simulink model "rfsoc4x2_ospfb_128"  (R2021a)
settings: Solver=VariableStepAuto  StartTime=0.0  StopTime=2048  RelTol=1e-3
undefined symbols (not defined in the file): pfb_coeff_gen_calc
libraries: xbsIndex_r4 x25898, casper_library_delays x113, casper_library_misc x68, xps_library x1
(part 5 of 221)

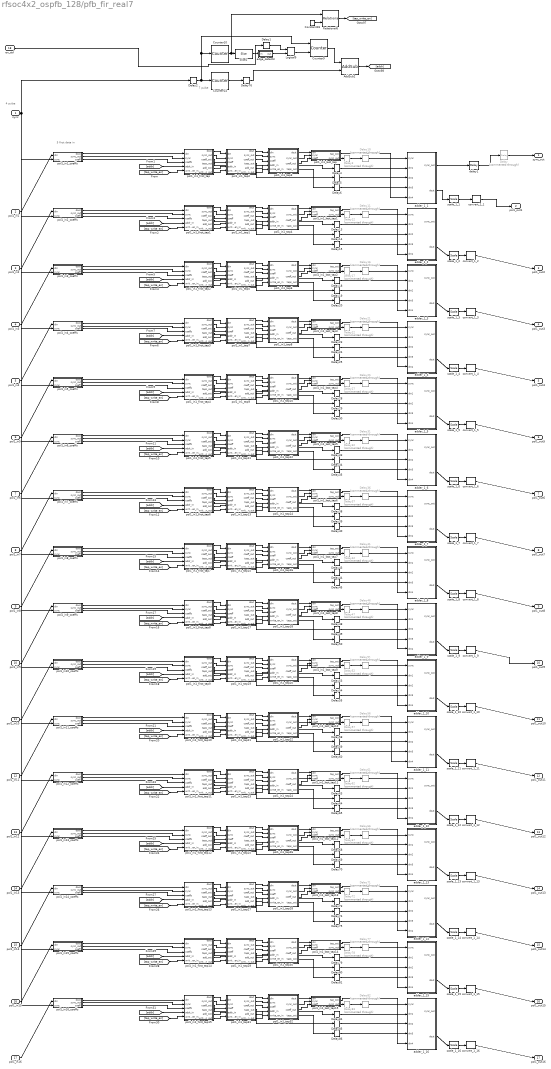
== system rfsoc4x2_ospfb_128/pfb_fir_real7 ==
  note: 5 first data in
  note: 7 pulse
  note: 4 pulse
  sync : Inport
  pol1_in1 : Inport  Port=2
  pol1_in2 : Inport  Port=3
  pol1_in3 : Inport  Port=4
  pol1_in4 : Inport  Port=5
  pol1_in5 : Inport  Port=6
  pol1_in6 : Inport  Port=7
  pol1_in7 : Inport  Port=8
  pol1_in8 : Inport  Port=9
  pol1_in9 : Inport  Port=10
  pol1_in10 : Inport  Port=11
  pol1_in11 : Inport  Port=12
  pol1_in12 : Inport  Port=13
  pol1_in13 : Inport  Port=14
  pol1_in14 : Inport  Port=15
  pol1_in15 : Inport  Port=16
  pol1_in16 : Inport  Port=17
  en_ctrl : Inport  Port=18
  AddSub2 : xbsIndex_r4/AddSub  mode=Addition  use_carryin=off  use_carryout=off  en=off  latency=0  precision=User Defined  arith_type=Unsigned  n_bits=5-1  bin_pt=0  quantization=Truncate  overflow=Wrap  use_behavioral_HDL=off  hw_selection=Fabric  pipelined=off  dbl_ovrd=off  block_type=addsub
  Constant28 : xbsIndex_r4/Constant  const=7  gui_display_data_type=Fixed-point  arith_type=Unsigned  n_bits=log2((2^8 / 2^4))  bin_pt=0  preci_type=Single  exp_width=8  frac_width=24  explicit_period=off  period=1  equ=P=C  opselect=C  inp2=PCIN>>17  opr=+  inp1=P  carry=CIN  dbl_ovrd=off  block_type=constant
  Counter10 : xbsIndex_r4/Counter  cnt_type=Free Running  cnt_to=Inf  operation=Up  start_count=16/2  cnt_by_val=1  arith_type=Unsigned  n_bits=5-1  bin_pt=0  load_pin=off  rst=on  en=off  explicit_period=on  period=1  use_behavioral_HDL=off  implementation=Fabric  dbl_ovrd=off  block_type=counter
  Counter14 : xbsIndex_r4/Counter  cnt_type=Free Running  cnt_to=1023  operation=Up  start_count=0  cnt_by_val=1  arith_type=Unsigned  n_bits=4-1  bin_pt=0  load_pin=off  rst=on  en=off  explicit_period=on  period=1  use_behavioral_HDL=off  implementation=Fabric  dbl_ovrd=off  block_type=counter
  Counter9 : xbsIndex_r4/Counter  cnt_type=Free Running  cnt_to=0  operation=Up  start_count=0  cnt_by_val=16/2  arith_type=Unsigned  n_bits=5-1  bin_pt=0  load_pin=off  rst=on  en=on  explicit_period=on  period=1  use_behavioral_HDL=off  implementation=Fabric  dbl_ovrd=off  block_type=counter
  Delay : xbsIndex_r4/Delay  Commented=through  rst=off  infoeditControl=Selection of Reset will increase slice count due to use of real FFs and instead of SRLs  en=off  latency=47  reg_retiming=off  dbl_ovrd=off  block_type=delay
  Delay1 : xbsIndex_r4/Delay  rst=off  infoeditControl=Selection of Reset will increase slice count due to use of real FFs and instead of SRLs  en=off  latency=4  reg_retiming=off  dbl_ovrd=off  block_type=delay
  Delay{10..11,16,21,26,31,36,41,46,51,56,61,66,71,77,82} (16 alike) : xbsIndex_r4/Delay  Commented=through  rst=off  infoeditControl=Selection of Reset will increase slice count due to use of real FFs and instead of SRLs  en=off  latency=2  reg_retiming=off  dbl_ovrd=off  block_type=delay
  Delay{3,12,17,22,27,32,37,42,47,52,57,62,67,72,78,83} (16 alike) : xbsIndex_r4/Delay  Commented=through  rst=off  infoeditControl=Selection of Reset will increase slice count due to use of real FFs and instead of SRLs  en=off  latency=3  reg_retiming=off  dbl_ovrd=off  block_type=delay
  Delay{2,4,13,18,23,28,33,38,43,48,53,58,63,68,73,79,84} (17 alike) : xbsIndex_r4/Delay  rst=off  infoeditControl=Selection of Reset will increase slice count due to use of real FFs and instead of SRLs  en=off  latency=3  reg_retiming=off  dbl_ovrd=off  block_type=delay
  Delay{5,14,19,24,29,34,39,44,49,54,59,64,69,74,80,85} (16 alike) : xbsIndex_r4/Delay  rst=off  infoeditControl=Selection of Reset will increase slice count due to use of real FFs and instead of SRLs  en=off  latency=2  reg_retiming=off  dbl_ovrd=off  block_type=delay
  Delay{6,15,20,25,30,35,40,45,50,55,60,65,70,75..76,81,86} (17 alike) : xbsIndex_r4/Delay  rst=off  infoeditControl=Selection of Reset will increase slice count due to use of real FFs and instead of SRLs  en=off  latency=1  reg_retiming=off  dbl_ovrd=off  block_type=delay
  Logical9 : xbsIndex_r4/Logical  logical_function=AND  inputs=2  en=off  latency=0  precision=Full  arith_type=Unsigned  n_bits=16  bin_pt=0  align_bp=on  dbl_ovrd=off  block_type=logical
  Relational6 : xbsIndex_r4/Relational  mode=a>b  op_type=Bool  en=off  latency=1  dbl_ovrd=off  block_type=relational
  Slice2 : xbsIndex_r4/Slice  nbits=1  boolean_output=on  mode=Upper Bit Location + Width  bit1=0  base1=MSB of Input  bit0=0  base0=LSB of Input  dbl_ovrd=off  block_type=slice
  adder_1_1 : Subsystem  AncestorBlock=casper_library_misc/adder_tree  mask(adder_tree){n_inputs=4, csp_latency=1, adder_imp=Fabric, first_stage_hdl=on, floating_point=off, dvalid_en=off, float_type=single, frac_width=0, exp_width=0}
      mask prompts: n_inputs "Number of Inputs"; csp_latency "Add Latency"; adder_imp "Adder implementation"; first_stage_hdl "Use behavioural HDL for first stage of adders"; floating_point "floating point"; float_type "float type"; frac_width "fraction length"; exp_width "exponent length"
      mask help:
      | Sums all inputs using a tree of adds and delays.
      |
      | Number of inputs: The number of inputs to the block to be summed
      | Add latency: The number of clock cycles to perform one addition (affects timing)..
      | Adder implementation: choice of fabric or DSP48E core, or behavioral HDL
      | Use behavioural HDL for first stage of adders: Causes the first stage of adders to be absorbed into DSP blocks if multipliers precede them (Virtex 5). Overrides Adder implementation
      mask init:
      | adder_tree_init(gcb, ...
      |     'n_inputs', n_inputs, ...
      |     'csp_latency', csp_latency, ...
      |     'adder_imp', adder_imp, ...
      |     'dvalid_en', dvalid_en, ...
      |     'floating_point', floating_point, ...
      |     'float_type', float_type, ...
      |     'exp_width', exp_width, ...
      |     'frac_width', frac_width, ...     
      |     'first_stage_hdl', first_stage_hdl);
      settings: AttributesFormatString=latency 2
      mask Help: eval('xlWeb(''http://casper.berkeley.edu/wiki/Adder_tree'')')
      mask TypeOptions adder_imp: Behavioral | Fabric | DSP48
      mask Callback floating_point:
      | onoff = get_param(gcb, 'floating_point');
      | if strcmp(onoff,'on')
      |     enable_fixpt = 'off';
      |     set_param_state(gcb, 'float_type', 'on')
      | 
      |     f_type = get_param(gcb, 'float_type');
      |     if strcmp(f_type,'custom')
      |         set_param_state(gcb, 'exp_width', 'on')
      |         set_param_state(gcb, 'frac_width', 'on')
      |     else
      |         set_param_state(gcb, 'exp_width', 'off')
      |         set_param_state(gcb, 'frac_width', 'off')
      |     end
      | 
      | 
      | else
      |     enable_fixpt = 'on';
      |     set_param_state(gcb, 'float_type', 'off')
      |     set_param_state(gcb, 'exp_width', 'off')
      |     set_param_state(gcb, 'frac_width', 'off')
      | end
      mask TypeOptions float_type: single | custom
      mask Callback float_type:
      | f_type = get_param(gcb, 'float_type');
      | if strcmp(f_type,'custom')
      |     set_param_state(gcb, 'exp_width', 'on')
      |     set_param_state(gcb, 'frac_width', 'on')
      | else
      |     set_param_state(gcb, 'exp_width', 'off')
      |     set_param_state(gcb, 'frac_width', 'off')
      | end
  adder_1_10 : Subsystem  AncestorBlock=casper_library_misc/adder_tree  mask(adder_tree){n_inputs=4, csp_latency=1, adder_imp=Fabric, first_stage_hdl=on, floating_point=off, dvalid_en=off, float_type=single, frac_width=0, exp_width=0}
      mask prompts: n_inputs "Number of Inputs"; csp_latency "Add Latency"; adder_imp "Adder implementation"; first_stage_hdl "Use behavioural HDL for first stage of adders"; floating_point "floating point"; float_type "float type"; frac_width "fraction length"; exp_width "exponent length"
      mask help:
      | Sums all inputs using a tree of adds and delays.
      |
      | Number of inputs: The number of inputs to the block to be summed
      | Add latency: The number of clock cycles to perform one addition (affects timing)..
      | Adder implementation: choice of fabric or DSP48E core, or behavioral HDL
      | Use behavioural HDL for first stage of adders: Causes the first stage of adders to be absorbed into DSP blocks if multipliers precede them (Virtex 5). Overrides Adder implementation
      mask init: same as rfsoc4x2_ospfb_128/pfb_fir_real7/adder_1_1
      settings: AttributesFormatString=latency 2
      mask Help: eval('xlWeb(''http://casper.berkeley.edu/wiki/Adder_tree'')')
      mask TypeOptions adder_imp: Behavioral | Fabric | DSP48
      mask Callback floating_point:
      | onoff = get_param(gcb, 'floating_point');
      | if strcmp(onoff,'on')
      |     enable_fixpt = 'off';
      |     set_param_state(gcb, 'float_type', 'on')
      | 
      |     f_type = get_param(gcb, 'float_type');
      |     if strcmp(f_type,'custom')
      |         set_param_state(gcb, 'exp_width', 'on')
      |         set_param_state(gcb, 'frac_width', 'on')
      |     else
      |         set_param_state(gcb, 'exp_width', 'off')
      |         set_param_state(gcb, 'frac_width', 'off')
      |     end
      | 
      | 
      | else
      |     enable_fixpt = 'on';
      |     set_param_state(gcb, 'float_type', 'off')
      |     set_param_state(gcb, 'exp_width', 'off')
      |     set_param_state(gcb, 'frac_width', 'off')
      | end
      mask TypeOptions float_type: single | custom
      mask Callback float_type:
      | f_type = get_param(gcb, 'float_type');
      | if strcmp(f_type,'custom')
      |     set_param_state(gcb, 'exp_width', 'on')
      |     set_param_state(gcb, 'frac_width', 'on')
      | else
      |     set_param_state(gcb, 'exp_width', 'off')
      |     set_param_state(gcb, 'frac_width', 'off')
      | end
  adder_1_11 : Subsystem  AncestorBlock=casper_library_misc/adder_tree  mask(adder_tree){n_inputs=4, csp_latency=1, adder_imp=Fabric, first_stage_hdl=on, floating_point=off, dvalid_en=off, float_type=single, frac_width=0, exp_width=0}
      mask prompts: n_inputs "Number of Inputs"; csp_latency "Add Latency"; adder_imp "Adder implementation"; first_stage_hdl "Use behavioural HDL for first stage of adders"; floating_point "floating point"; float_type "float type"; frac_width "fraction length"; exp_width "exponent length"
      mask help:
      | Sums all inputs using a tree of adds and delays.
      |
      | Number of inputs: The number of inputs to the block to be summed
      | Add latency: The number of clock cycles to perform one addition (affects timing)..
      | Adder implementation: choice of fabric or DSP48E core, or behavioral HDL
      | Use behavioural HDL for first stage of adders: Causes the first stage of adders to be absorbed into DSP blocks if multipliers precede them (Virtex 5). Overrides Adder implementation
      mask init: same as rfsoc4x2_ospfb_128/pfb_fir_real7/adder_1_1
      settings: AttributesFormatString=latency 2
      mask Help: eval('xlWeb(''http://casper.berkeley.edu/wiki/Adder_tree'')')
      mask TypeOptions adder_imp: Behavioral | Fabric | DSP48
      mask Callback floating_point:
      | onoff = get_param(gcb, 'floating_point');
      | if strcmp(onoff,'on')
      |     enable_fixpt = 'off';
      |     set_param_state(gcb, 'float_type', 'on')
      | 
      |     f_type = get_param(gcb, 'float_type');
      |     if strcmp(f_type,'custom')
      |         set_param_state(gcb, 'exp_width', 'on')
      |         set_param_state(gcb, 'frac_width', 'on')
      |     else
      |         set_param_state(gcb, 'exp_width', 'off')
      |         set_param_state(gcb, 'frac_width', 'off')
      |     end
      | 
      | 
      | else
      |     enable_fixpt = 'on';
      |     set_param_state(gcb, 'float_type', 'off')
      |     set_param_state(gcb, 'exp_width', 'off')
      |     set_param_state(gcb, 'frac_width', 'off')
      | end
      mask TypeOptions float_type: single | custom
      mask Callback float_type:
      | f_type = get_param(gcb, 'float_type');
      | if strcmp(f_type,'custom')
      |     set_param_state(gcb, 'exp_width', 'on')
      |     set_param_state(gcb, 'frac_width', 'on')
      | else
      |     set_param_state(gcb, 'exp_width', 'off')
      |     set_param_state(gcb, 'frac_width', 'off')
      | end
  adder_1_12 : Subsystem  AncestorBlock=casper_library_misc/adder_tree  mask(adder_tree){n_inputs=4, csp_latency=1, adder_imp=Fabric, first_stage_hdl=on, floating_point=off, dvalid_en=off, float_type=single, frac_width=0, exp_width=0}
      mask prompts: n_inputs "Number of Inputs"; csp_latency "Add Latency"; adder_imp "Adder implementation"; first_stage_hdl "Use behavioural HDL for first stage of adders"; floating_point "floating point"; float_type "float type"; frac_width "fraction length"; exp_width "exponent length"
      mask help:
      | Sums all inputs using a tree of adds and delays.
      |
      | Number of inputs: The number of inputs to the block to be summed
      | Add latency: The number of clock cycles to perform one addition (affects timing)..
      | Adder implementation: choice of fabric or DSP48E core, or behavioral HDL
      | Use behavioural HDL for first stage of adders: Causes the first stage of adders to be absorbed into DSP blocks if multipliers precede them (Virtex 5). Overrides Adder implementation
      mask init: same as rfsoc4x2_ospfb_128/pfb_fir_real7/adder_1_1
      settings: AttributesFormatString=latency 2
      mask Help: eval('xlWeb(''http://casper.berkeley.edu/wiki/Adder_tree'')')
      mask TypeOptions adder_imp: Behavioral | Fabric | DSP48
      mask Callback floating_point:
      | onoff = get_param(gcb, 'floating_point');
      | if strcmp(onoff,'on')
      |     enable_fixpt = 'off';
      |     set_param_state(gcb, 'float_type', 'on')
      | 
      |     f_type = get_param(gcb, 'float_type');
      |     if strcmp(f_type,'custom')
      |         set_param_state(gcb, 'exp_width', 'on')
      |         set_param_state(gcb, 'frac_width', 'on')
      |     else
      |         set_param_state(gcb, 'exp_width', 'off')
      |         set_param_state(gcb, 'frac_width', 'off')
      |     end
      | 
      | 
      | else
      |     enable_fixpt = 'on';
      |     set_param_state(gcb, 'float_type', 'off')
      |     set_param_state(gcb, 'exp_width', 'off')
      |     set_param_state(gcb, 'frac_width', 'off')
      | end
      mask TypeOptions float_type: single | custom
      mask Callback float_type:
      | f_type = get_param(gcb, 'float_type');
      | if strcmp(f_type,'custom')
      |     set_param_state(gcb, 'exp_width', 'on')
      |     set_param_state(gcb, 'frac_width', 'on')
      | else
      |     set_param_state(gcb, 'exp_width', 'off')
      |     set_param_state(gcb, 'frac_width', 'off')
      | end
  adder_1_13 : Subsystem  AncestorBlock=casper_library_misc/adder_tree  mask(adder_tree){n_inputs=4, csp_latency=1, adder_imp=Fabric, first_stage_hdl=on, floating_point=off, dvalid_en=off, float_type=single, frac_width=0, exp_width=0}
      mask prompts: n_inputs "Number of Inputs"; csp_latency "Add Latency"; adder_imp "Adder implementation"; first_stage_hdl "Use behavioural HDL for first stage of adders"; floating_point "floating point"; float_type "float type"; frac_width "fraction length"; exp_width "exponent length"
      mask help:
      | Sums all inputs using a tree of adds and delays.
      |
      | Number of inputs: The number of inputs to the block to be summed
      | Add latency: The number of clock cycles to perform one addition (affects timing)..
      | Adder implementation: choice of fabric or DSP48E core, or behavioral HDL
      | Use behavioural HDL for first stage of adders: Causes the first stage of adders to be absorbed into DSP blocks if multipliers precede them (Virtex 5). Overrides Adder implementation
      mask init: same as rfsoc4x2_ospfb_128/pfb_fir_real7/adder_1_1
      settings: AttributesFormatString=latency 2
      mask Help: eval('xlWeb(''http://casper.berkeley.edu/wiki/Adder_tree'')')
      mask TypeOptions adder_imp: Behavioral | Fabric | DSP48
      mask Callback floating_point:
      | onoff = get_param(gcb, 'floating_point');
      | if strcmp(onoff,'on')
      |     enable_fixpt = 'off';
      |     set_param_state(gcb, 'float_type', 'on')
      | 
      |     f_type = get_param(gcb, 'float_type');
      |     if strcmp(f_type,'custom')
      |         set_param_state(gcb, 'exp_width', 'on')
      |         set_param_state(gcb, 'frac_width', 'on')
      |     else
      |         set_param_state(gcb, 'exp_width', 'off')
      |         set_param_state(gcb, 'frac_width', 'off')
      |     end
      | 
      | 
      | else
      |     enable_fixpt = 'on';
      |     set_param_state(gcb, 'float_type', 'off')
      |     set_param_state(gcb, 'exp_width', 'off')
      |     set_param_state(gcb, 'frac_width', 'off')
      | end
      mask TypeOptions float_type: single | custom
      mask Callback float_type:
      | f_type = get_param(gcb, 'float_type');
      | if strcmp(f_type,'custom')
      |     set_param_state(gcb, 'exp_width', 'on')
      |     set_param_state(gcb, 'frac_width', 'on')
      | else
      |     set_param_state(gcb, 'exp_width', 'off')
      |     set_param_state(gcb, 'frac_width', 'off')
      | end
  adder_1_14 : Subsystem  AncestorBlock=casper_library_misc/adder_tree  mask(adder_tree){n_inputs=4, csp_latency=1, adder_imp=Fabric, first_stage_hdl=on, floating_point=off, dvalid_en=off, float_type=single, frac_width=0, exp_width=0}
      mask prompts: n_inputs "Number of Inputs"; csp_latency "Add Latency"; adder_imp "Adder implementation"; first_stage_hdl "Use behavioural HDL for first stage of adders"; floating_point "floating point"; float_type "float type"; frac_width "fraction length"; exp_width "exponent length"
      mask help:
      | Sums all inputs using a tree of adds and delays.
      |
      | Number of inputs: The number of inputs to the block to be summed
      | Add latency: The number of clock cycles to perform one addition (affects timing)..
      | Adder implementation: choice of fabric or DSP48E core, or behavioral HDL
      | Use behavioural HDL for first stage of adders: Causes the first stage of adders to be absorbed into DSP blocks if multipliers precede them (Virtex 5). Overrides Adder implementation
      mask init: same as rfsoc4x2_ospfb_128/pfb_fir_real7/adder_1_1
      settings: AttributesFormatString=latency 2
      mask Help: eval('xlWeb(''http://casper.berkeley.edu/wiki/Adder_tree'')')
      mask TypeOptions adder_imp: Behavioral | Fabric | DSP48
      mask Callback floating_point:
      | onoff = get_param(gcb, 'floating_point');
      | if strcmp(onoff,'on')
      |     enable_fixpt = 'off';
      |     set_param_state(gcb, 'float_type', 'on')
      | 
      |     f_type = get_param(gcb, 'float_type');
      |     if strcmp(f_type,'custom')
      |         set_param_state(gcb, 'exp_width', 'on')
      |         set_param_state(gcb, 'frac_width', 'on')
      |     else
      |         set_param_state(gcb, 'exp_width', 'off')
      |         set_param_state(gcb, 'frac_width', 'off')
      |     end
      | 
      | 
      | else
      |     enable_fixpt = 'on';
      |     set_param_state(gcb, 'float_type', 'off')
      |     set_param_state(gcb, 'exp_width', 'off')
      |     set_param_state(gcb, 'frac_width', 'off')
      | end
      mask TypeOptions float_type: single | custom
      mask Callback float_type:
      | f_type = get_param(gcb, 'float_type');
      | if strcmp(f_type,'custom')
      |     set_param_state(gcb, 'exp_width', 'on')
      |     set_param_state(gcb, 'frac_width', 'on')
      | else
      |     set_param_state(gcb, 'exp_width', 'off')
      |     set_param_state(gcb, 'frac_width', 'off')
      | end
  adder_1_15 : Subsystem  AncestorBlock=casper_library_misc/adder_tree  mask(adder_tree){n_inputs=4, csp_latency=1, adder_imp=Fabric, first_stage_hdl=on, floating_point=off, dvalid_en=off, float_type=single, frac_width=0, exp_width=0}
      mask prompts: n_inputs "Number of Inputs"; csp_latency "Add Latency"; adder_imp "Adder implementation"; first_stage_hdl "Use behavioural HDL for first stage of adders"; floating_point "floating point"; float_type "float type"; frac_width "fraction length"; exp_width "exponent length"
      mask help:
      | Sums all inputs using a tree of adds and delays.
      |
      | Number of inputs: The number of inputs to the block to be summed
      | Add latency: The number of clock cycles to perform one addition (affects timing)..
      | Adder implementation: choice of fabric or DSP48E core, or behavioral HDL
      | Use behavioural HDL for first stage of adders: Causes the first stage of adders to be absorbed into DSP blocks if multipliers precede them (Virtex 5). Overrides Adder implementation
      mask init: same as rfsoc4x2_ospfb_128/pfb_fir_real7/adder_1_1
      settings: AttributesFormatString=latency 2
      mask Help: eval('xlWeb(''http://casper.berkeley.edu/wiki/Adder_tree'')')
      mask TypeOptions adder_imp: Behavioral | Fabric | DSP48
      mask Callback floating_point:
      | onoff = get_param(gcb, 'floating_point');
      | if strcmp(onoff,'on')
      |     enable_fixpt = 'off';
      |     set_param_state(gcb, 'float_type', 'on')
      | 
      |     f_type = get_param(gcb, 'float_type');
      |     if strcmp(f_type,'custom')
      |         set_param_state(gcb, 'exp_width', 'on')
      |         set_param_state(gcb, 'frac_width', 'on')
      |     else
      |         set_param_state(gcb, 'exp_width', 'off')
      |         set_param_state(gcb, 'frac_width', 'off')
      |     end
      | 
      | 
      | else
      |     enable_fixpt = 'on';
      |     set_param_state(gcb, 'float_type', 'off')
      |     set_param_state(gcb, 'exp_width', 'off')
      |     set_param_state(gcb, 'frac_width', 'off')
      | end
      mask TypeOptions float_type: single | custom
      mask Callback float_type:
      | f_type = get_param(gcb, 'float_type');
      | if strcmp(f_type,'custom')
      |     set_param_state(gcb, 'exp_width', 'on')
      |     set_param_state(gcb, 'frac_width', 'on')
      | else
      |     set_param_state(gcb, 'exp_width', 'off')
      |     set_param_state(gcb, 'frac_width', 'off')
      | end
  adder_1_16 : Subsystem  AncestorBlock=casper_library_misc/adder_tree  mask(adder_tree){n_inputs=4, csp_latency=1, adder_imp=Fabric, first_stage_hdl=on, floating_point=off, dvalid_en=off, float_type=single, frac_width=0, exp_width=0}
      mask prompts: n_inputs "Number of Inputs"; csp_latency "Add Latency"; adder_imp "Adder implementation"; first_stage_hdl "Use behavioural HDL for first stage of adders"; floating_point "floating point"; float_type "float type"; frac_width "fraction length"; exp_width "exponent length"
      mask help:
      | Sums all inputs using a tree of adds and delays.
      |
      | Number of inputs: The number of inputs to the block to be summed
      | Add latency: The number of clock cycles to perform one addition (affects timing)..
      | Adder implementation: choice of fabric or DSP48E core, or behavioral HDL
      | Use behavioural HDL for first stage of adders: Causes the first stage of adders to be absorbed into DSP blocks if multipliers precede them (Virtex 5). Overrides Adder implementation
      mask init: same as rfsoc4x2_ospfb_128/pfb_fir_real7/adder_1_1
      settings: AttributesFormatString=latency 2
      mask Help: eval('xlWeb(''http://casper.berkeley.edu/wiki/Adder_tree'')')
      mask TypeOptions adder_imp: Behavioral | Fabric | DSP48
      mask Callback floating_point:
      | onoff = get_param(gcb, 'floating_point');
      | if strcmp(onoff,'on')
      |     enable_fixpt = 'off';
      |     set_param_state(gcb, 'float_type', 'on')
      | 
      |     f_type = get_param(gcb, 'float_type');
      |     if strcmp(f_type,'custom')
      |         set_param_state(gcb, 'exp_width', 'on')
      |         set_param_state(gcb, 'frac_width', 'on')
      |     else
      |         set_param_state(gcb, 'exp_width', 'off')
      |         set_param_state(gcb, 'frac_width', 'off')
      |     end
      | 
      | 
      | else
      |     enable_fixpt = 'on';
      |     set_param_state(gcb, 'float_type', 'off')
      |     set_param_state(gcb, 'exp_width', 'off')
      |     set_param_state(gcb, 'frac_width', 'off')
      | end
      mask TypeOptions float_type: single | custom
      mask Callback float_type:
      | f_type = get_param(gcb, 'float_type');
      | if strcmp(f_type,'custom')
      |     set_param_state(gcb, 'exp_width', 'on')
      |     set_param_state(gcb, 'frac_width', 'on')
      | else
      |     set_param_state(gcb, 'exp_width', 'off')
      |     set_param_state(gcb, 'frac_width', 'off')
      | end
  adder_1_2 : Subsystem  AncestorBlock=casper_library_misc/adder_tree  mask(adder_tree){n_inputs=4, csp_latency=1, adder_imp=Fabric, first_stage_hdl=on, floating_point=off, dvalid_en=off, float_type=single, frac_width=0, exp_width=0}
      mask prompts: n_inputs "Number of Inputs"; csp_latency "Add Latency"; adder_imp "Adder implementation"; first_stage_hdl "Use behavioural HDL for first stage of adders"; floating_point "floating point"; float_type "float type"; frac_width "fraction length"; exp_width "exponent length"
      mask help:
      | Sums all inputs using a tree of adds and delays.
      |
      | Number of inputs: The number of inputs to the block to be summed
      | Add latency: The number of clock cycles to perform one addition (affects timing)..
      | Adder implementation: choice of fabric or DSP48E core, or behavioral HDL
      | Use behavioural HDL for first stage of adders: Causes the first stage of adders to be absorbed into DSP blocks if multipliers precede them (Virtex 5). Overrides Adder implementation
      mask init: same as rfsoc4x2_ospfb_128/pfb_fir_real7/adder_1_1
      settings: AttributesFormatString=latency 2
      mask Help: eval('xlWeb(''http://casper.berkeley.edu/wiki/Adder_tree'')')
      mask TypeOptions adder_imp: Behavioral | Fabric | DSP48
      mask Callback floating_point:
      | onoff = get_param(gcb, 'floating_point');
      | if strcmp(onoff,'on')
      |     enable_fixpt = 'off';
      |     set_param_state(gcb, 'float_type', 'on')
      | 
      |     f_type = get_param(gcb, 'float_type');
      |     if strcmp(f_type,'custom')
      |         set_param_state(gcb, 'exp_width', 'on')
      |         set_param_state(gcb, 'frac_width', 'on')
      |     else
      |         set_param_state(gcb, 'exp_width', 'off')
      |         set_param_state(gcb, 'frac_width', 'off')
      |     end
      | 
      | 
      | else
      |     enable_fixpt = 'on';
      |     set_param_state(gcb, 'float_type', 'off')
      |     set_param_state(gcb, 'exp_width', 'off')
      |     set_param_state(gcb, 'frac_width', 'off')
      | end
      mask TypeOptions float_type: single | custom
      mask Callback float_type:
      | f_type = get_param(gcb, 'float_type');
      | if strcmp(f_type,'custom')
      |     set_param_state(gcb, 'exp_width', 'on')
      |     set_param_state(gcb, 'frac_width', 'on')
      | else
      |     set_param_state(gcb, 'exp_width', 'off')
      |     set_param_state(gcb, 'frac_width', 'off')
      | end
  adder_1_3 : Subsystem  AncestorBlock=casper_library_misc/adder_tree  mask(adder_tree){n_inputs=4, csp_latency=1, adder_imp=Fabric, first_stage_hdl=on, floating_point=off, dvalid_en=off, float_type=single, frac_width=0, exp_width=0}
      mask prompts: n_inputs "Number of Inputs"; csp_latency "Add Latency"; adder_imp "Adder implementation"; first_stage_hdl "Use behavioural HDL for first stage of adders"; floating_point "floating point"; float_type "float type"; frac_width "fraction length"; exp_width "exponent length"
      mask help:
      | Sums all inputs using a tree of adds and delays.
      |
      | Number of inputs: The number of inputs to the block to be summed
      | Add latency: The number of clock cycles to perform one addition (affects timing)..
      | Adder implementation: choice of fabric or DSP48E core, or behavioral HDL
      | Use behavioural HDL for first stage of adders: Causes the first stage of adders to be absorbed into DSP blocks if multipliers precede them (Virtex 5). Overrides Adder implementation
      mask init: same as rfsoc4x2_ospfb_128/pfb_fir_real7/adder_1_1
      settings: AttributesFormatString=latency 2
      mask Help: eval('xlWeb(''http://casper.berkeley.edu/wiki/Adder_tree'')')
      mask TypeOptions adder_imp: Behavioral | Fabric | DSP48
      mask Callback floating_point:
      | onoff = get_param(gcb, 'floating_point');
      | if strcmp(onoff,'on')
      |     enable_fixpt = 'off';
      |     set_param_state(gcb, 'float_type', 'on')
      | 
      |     f_type = get_param(gcb, 'float_type');
      |     if strcmp(f_type,'custom')
      |         set_param_state(gcb, 'exp_width', 'on')
      |         set_param_state(gcb, 'frac_width', 'on')
      |     else
      |         set_param_state(gcb, 'exp_width', 'off')
      |         set_param_state(gcb, 'frac_width', 'off')
      |     end
      | 
      | 
      | else
      |     enable_fixpt = 'on';
      |     set_param_state(gcb, 'float_type', 'off')
      |     set_param_state(gcb, 'exp_width', 'off')
      |     set_param_state(gcb, 'frac_width', 'off')
      | end
      mask TypeOptions float_type: single | custom
      mask Callback float_type:
      | f_type = get_param(gcb, 'float_type');
      | if strcmp(f_type,'custom')
      |     set_param_state(gcb, 'exp_width', 'on')
      |     set_param_state(gcb, 'frac_width', 'on')
      | else
      |     set_param_state(gcb, 'exp_width', 'off')
      |     set_param_state(gcb, 'frac_width', 'off')
      | end
  adder_1_4 : Subsystem  AncestorBlock=casper_library_misc/adder_tree  mask(adder_tree){n_inputs=4, csp_latency=1, adder_imp=Fabric, first_stage_hdl=on, floating_point=off, dvalid_en=off, float_type=single, frac_width=0, exp_width=0}
      mask prompts: n_inputs "Number of Inputs"; csp_latency "Add Latency"; adder_imp "Adder implementation"; first_stage_hdl "Use behavioural HDL for first stage of adders"; floating_point "floating point"; float_type "float type"; frac_width "fraction length"; exp_width "exponent length"
      mask help:
      | Sums all inputs using a tree of adds and delays.
      |
      | Number of inputs: The number of inputs to the block to be summed
      | Add latency: The number of clock cycles to perform one addition (affects timing)..
      | Adder implementation: choice of fabric or DSP48E core, or behavioral HDL
      | Use behavioural HDL for first stage of adders: Causes the first stage of adders to be absorbed into DSP blocks if multipliers precede them (Virtex 5). Overrides Adder implementation
      mask init: same as rfsoc4x2_ospfb_128/pfb_fir_real7/adder_1_1
      settings: AttributesFormatString=latency 2
      mask Help: eval('xlWeb(''http://casper.berkeley.edu/wiki/Adder_tree'')')
      mask TypeOptions adder_imp: Behavioral | Fabric | DSP48
      mask Callback floating_point:
      | onoff = get_param(gcb, 'floating_point');
      | if strcmp(onoff,'on')
      |     enable_fixpt = 'off';
      |     set_param_state(gcb, 'float_type', 'on')
      | 
      |     f_type = get_param(gcb, 'float_type');
      |     if strcmp(f_type,'custom')
      |         set_param_state(gcb, 'exp_width', 'on')
      |         set_param_state(gcb, 'frac_width', 'on')
      |     else
      |         set_param_state(gcb, 'exp_width', 'off')
      |         set_param_state(gcb, 'frac_width', 'off')
      |     end
      | 
      | 
      | else
      |     enable_fixpt = 'on';
      |     set_param_state(gcb, 'float_type', 'off')
      |     set_param_state(gcb, 'exp_width', 'off')
      |     set_param_state(gcb, 'frac_width', 'off')
      | end
      mask TypeOptions float_type: single | custom
      mask Callback float_type:
      | f_type = get_param(gcb, 'float_type');
      | if strcmp(f_type,'custom')
      |     set_param_state(gcb, 'exp_width', 'on')
      |     set_param_state(gcb, 'frac_width', 'on')
      | else
      |     set_param_state(gcb, 'exp_width', 'off')
      |     set_param_state(gcb, 'frac_width', 'off')
      | end
  adder_1_5 : Subsystem  AncestorBlock=casper_library_misc/adder_tree  mask(adder_tree){n_inputs=4, csp_latency=1, adder_imp=Fabric, first_stage_hdl=on, floating_point=off, dvalid_en=off, float_type=single, frac_width=0, exp_width=0}
      mask prompts: n_inputs "Number of Inputs"; csp_latency "Add Latency"; adder_imp "Adder implementation"; first_stage_hdl "Use behavioural HDL for first stage of adders"; floating_point "floating point"; float_type "float type"; frac_width "fraction length"; exp_width "exponent length"
      mask help:
      | Sums all inputs using a tree of adds and delays.
      |
      | Number of inputs: The number of inputs to the block to be summed
      | Add latency: The number of clock cycles to perform one addition (affects timing)..
      | Adder implementation: choice of fabric or DSP48E core, or behavioral HDL
      | Use behavioural HDL for first stage of adders: Causes the first stage of adders to be absorbed into DSP blocks if multipliers precede them (Virtex 5). Overrides Adder implementation
      mask init: same as rfsoc4x2_ospfb_128/pfb_fir_real7/adder_1_1
      settings: AttributesFormatString=latency 2
      mask Help: eval('xlWeb(''http://casper.berkeley.edu/wiki/Adder_tree'')')
      mask TypeOptions adder_imp: Behavioral | Fabric | DSP48
      mask Callback floating_point:
      | onoff = get_param(gcb, 'floating_point');
      | if strcmp(onoff,'on')
      |     enable_fixpt = 'off';
      |     set_param_state(gcb, 'float_type', 'on')
      | 
      |     f_type = get_param(gcb, 'float_type');
      |     if strcmp(f_type,'custom')
      |         set_param_state(gcb, 'exp_width', 'on')
      |         set_param_state(gcb, 'frac_width', 'on')
      |     else
      |         set_param_state(gcb, 'exp_width', 'off')
      |         set_param_state(gcb, 'frac_width', 'off')
      |     end
      | 
      | 
      | else
      |     enable_fixpt = 'on';
      |     set_param_state(gcb, 'float_type', 'off')
      |     set_param_state(gcb, 'exp_width', 'off')
      |     set_param_state(gcb, 'frac_width', 'off')
      | end
      mask TypeOptions float_type: single | custom
      mask Callback float_type:
      | f_type = get_param(gcb, 'float_type');
      | if strcmp(f_type,'custom')
      |     set_param_state(gcb, 'exp_width', 'on')
      |     set_param_state(gcb, 'frac_width', 'on')
      | else
      |     set_param_state(gcb, 'exp_width', 'off')
      |     set_param_state(gcb, 'frac_width', 'off')
      | end
  adder_1_6 : Subsystem  AncestorBlock=casper_library_misc/adder_tree  mask(adder_tree){n_inputs=4, csp_latency=1, adder_imp=Fabric, first_stage_hdl=on, floating_point=off, dvalid_en=off, float_type=single, frac_width=0, exp_width=0}
      mask prompts: n_inputs "Number of Inputs"; csp_latency "Add Latency"; adder_imp "Adder implementation"; first_stage_hdl "Use behavioural HDL for first stage of adders"; floating_point "floating point"; float_type "float type"; frac_width "fraction length"; exp_width "exponent length"
      mask help:
      | Sums all inputs using a tree of adds and delays.
      |
      | Number of inputs: The number of inputs to the block to be summed
      | Add latency: The number of clock cycles to perform one addition (affects timing)..
      | Adder implementation: choice of fabric or DSP48E core, or behavioral HDL
      | Use behavioural HDL for first stage of adders: Causes the first stage of adders to be absorbed into DSP blocks if multipliers precede them (Virtex 5). Overrides Adder implementation
      mask init: same as rfsoc4x2_ospfb_128/pfb_fir_real7/adder_1_1
      settings: AttributesFormatString=latency 2
      mask Help: eval('xlWeb(''http://casper.berkeley.edu/wiki/Adder_tree'')')
      mask TypeOptions adder_imp: Behavioral | Fabric | DSP48
      mask Callback floating_point:
      | onoff = get_param(gcb, 'floating_point');
      | if strcmp(onoff,'on')
      |     enable_fixpt = 'off';
      |     set_param_state(gcb, 'float_type', 'on')
      | 
      |     f_type = get_param(gcb, 'float_type');
      |     if strcmp(f_type,'custom')
      |         set_param_state(gcb, 'exp_width', 'on')
      |         set_param_state(gcb, 'frac_width', 'on')
      |     else
      |         set_param_state(gcb, 'exp_width', 'off')
      |         set_param_state(gcb, 'frac_width', 'off')
      |     end
      | 
      | 
      | else
      |     enable_fixpt = 'on';
      |     set_param_state(gcb, 'float_type', 'off')
      |     set_param_state(gcb, 'exp_width', 'off')
      |     set_param_state(gcb, 'frac_width', 'off')
      | end
      mask TypeOptions float_type: single | custom
      mask Callback float_type:
      | f_type = get_param(gcb, 'float_type');
      | if strcmp(f_type,'custom')
      |     set_param_state(gcb, 'exp_width', 'on')
      |     set_param_state(gcb, 'frac_width', 'on')
      | else
      |     set_param_state(gcb, 'exp_width', 'off')
      |     set_param_state(gcb, 'frac_width', 'off')
      | end
  adder_1_7 : Subsystem  AncestorBlock=casper_library_misc/adder_tree  mask(adder_tree){n_inputs=4, csp_latency=1, adder_imp=Fabric, first_stage_hdl=on, floating_point=off, dvalid_en=off, float_type=single, frac_width=0, exp_width=0}
      mask prompts: n_inputs "Number of Inputs"; csp_latency "Add Latency"; adder_imp "Adder implementation"; first_stage_hdl "Use behavioural HDL for first stage of adders"; floating_point "floating point"; float_type "float type"; frac_width "fraction length"; exp_width "exponent length"
      mask help:
      | Sums all inputs using a tree of adds and delays.
      |
      | Number of inputs: The number of inputs to the block to be summed
      | Add latency: The number of clock cycles to perform one addition (affects timing)..
      | Adder implementation: choice of fabric or DSP48E core, or behavioral HDL
      | Use behavioural HDL for first stage of adders: Causes the first stage of adders to be absorbed into DSP blocks if multipliers precede them (Virtex 5). Overrides Adder implementation
      mask init: same as rfsoc4x2_ospfb_128/pfb_fir_real7/adder_1_1
      settings: AttributesFormatString=latency 2
      mask Help: eval('xlWeb(''http://casper.berkeley.edu/wiki/Adder_tree'')')
      mask TypeOptions adder_imp: Behavioral | Fabric | DSP48
      mask Callback floating_point:
      | onoff = get_param(gcb, 'floating_point');
      | if strcmp(onoff,'on')
      |     enable_fixpt = 'off';
      |     set_param_state(gcb, 'float_type', 'on')
      | 
      |     f_type = get_param(gcb, 'float_type');
      |     if strcmp(f_type,'custom')
      |         set_param_state(gcb, 'exp_width', 'on')
      |         set_param_state(gcb, 'frac_width', 'on')
      |     else
      |         set_param_state(gcb, 'exp_width', 'off')
      |         set_param_state(gcb, 'frac_width', 'off')
      |     end
      | 
      | 
      | else
      |     enable_fixpt = 'on';
      |     set_param_state(gcb, 'float_type', 'off')
      |     set_param_state(gcb, 'exp_width', 'off')
      |     set_param_state(gcb, 'frac_width', 'off')
      | end
      mask TypeOptions float_type: single | custom
      mask Callback float_type:
      | f_type = get_param(gcb, 'float_type');
      | if strcmp(f_type,'custom')
      |     set_param_state(gcb, 'exp_width', 'on')
      |     set_param_state(gcb, 'frac_width', 'on')
      | else
      |     set_param_state(gcb, 'exp_width', 'off')
      |     set_param_state(gcb, 'frac_width', 'off')
      | end
  adder_1_8 : Subsystem  AncestorBlock=casper_library_misc/adder_tree  mask(adder_tree){n_inputs=4, csp_latency=1, adder_imp=Fabric, first_stage_hdl=on, floating_point=off, dvalid_en=off, float_type=single, frac_width=0, exp_width=0}
      mask prompts: n_inputs "Number of Inputs"; csp_latency "Add Latency"; adder_imp "Adder implementation"; first_stage_hdl "Use behavioural HDL for first stage of adders"; floating_point "floating point"; float_type "float type"; frac_width "fraction length"; exp_width "exponent length"
      mask help:
      | Sums all inputs using a tree of adds and delays.
      |
      | Number of inputs: The number of inputs to the block to be summed
      | Add latency: The number of clock cycles to perform one addition (affects timing)..
      | Adder implementation: choice of fabric or DSP48E core, or behavioral HDL
      | Use behavioural HDL for first stage of adders: Causes the first stage of adders to be absorbed into DSP blocks if multipliers precede them (Virtex 5). Overrides Adder implementation
      mask init: same as rfsoc4x2_ospfb_128/pfb_fir_real7/adder_1_1
      settings: AttributesFormatString=latency 2
      mask Help: eval('xlWeb(''http://casper.berkeley.edu/wiki/Adder_tree'')')
      mask TypeOptions adder_imp: Behavioral | Fabric | DSP48
      mask Callback floating_point:
      | onoff = get_param(gcb, 'floating_point');
      | if strcmp(onoff,'on')
      |     enable_fixpt = 'off';
      |     set_param_state(gcb, 'float_type', 'on')
      | 
      |     f_type = get_param(gcb, 'float_type');
      |     if strcmp(f_type,'custom')
      |         set_param_state(gcb, 'exp_width', 'on')
      |         set_param_state(gcb, 'frac_width', 'on')
      |     else
      |         set_param_state(gcb, 'exp_width', 'off')
      |         set_param_state(gcb, 'frac_width', 'off')
      |     end
      | 
      | 
      | else
      |     enable_fixpt = 'on';
      |     set_param_state(gcb, 'float_type', 'off')
      |     set_param_state(gcb, 'exp_width', 'off')
      |     set_param_state(gcb, 'frac_width', 'off')
      | end
      mask TypeOptions float_type: single | custom
      mask Callback float_type:
      | f_type = get_param(gcb, 'float_type');
      | if strcmp(f_type,'custom')
      |     set_param_state(gcb, 'exp_width', 'on')
      |     set_param_state(gcb, 'frac_width', 'on')
      | else
      |     set_param_state(gcb, 'exp_width', 'off')
      |     set_param_state(gcb, 'frac_width', 'off')
      | end
  adder_1_9 : Subsystem  AncestorBlock=casper_library_misc/adder_tree  mask(adder_tree){n_inputs=4, csp_latency=1, adder_imp=Fabric, first_stage_hdl=on, floating_point=off, dvalid_en=off, float_type=single, frac_width=0, exp_width=0}
      mask prompts: n_inputs "Number of Inputs"; csp_latency "Add Latency"; adder_imp "Adder implementation"; first_stage_hdl "Use behavioural HDL for first stage of adders"; floating_point "floating point"; float_type "float type"; frac_width "fraction length"; exp_width "exponent length"
      mask help:
      | Sums all inputs using a tree of adds and delays.
      |
      | Number of inputs: The number of inputs to the block to be summed
      | Add latency: The number of clock cycles to perform one addition (affects timing)..
      | Adder implementation: choice of fabric or DSP48E core, or behavioral HDL
      | Use behavioural HDL for first stage of adders: Causes the first stage of adders to be absorbed into DSP blocks if multipliers precede them (Virtex 5). Overrides Adder implementation
      mask init: same as rfsoc4x2_ospfb_128/pfb_fir_real7/adder_1_1
      settings: AttributesFormatString=latency 2
      mask Help: eval('xlWeb(''http://casper.berkeley.edu/wiki/Adder_tree'')')
      mask TypeOptions adder_imp: Behavioral | Fabric | DSP48
      mask Callback floating_point:
      | onoff = get_param(gcb, 'floating_point');
      | if strcmp(onoff,'on')
      |     enable_fixpt = 'off';
      |     set_param_state(gcb, 'float_type', 'on')
      | 
      |     f_type = get_param(gcb, 'float_type');
      |     if strcmp(f_type,'custom')
      |         set_param_state(gcb, 'exp_width', 'on')
      |         set_param_state(gcb, 'frac_width', 'on')
      |     else
      |         set_param_state(gcb, 'exp_width', 'off')
      |         set_param_state(gcb, 'frac_width', 'off')
      |     end
      | 
      | 
      | else
      |     enable_fixpt = 'on';
      |     set_param_state(gcb, 'float_type', 'off')
      |     set_param_state(gcb, 'exp_width', 'off')
      |     set_param_state(gcb, 'frac_width', 'off')
      | end
      mask TypeOptions float_type: single | custom
      mask Callback float_type:
      | f_type = get_param(gcb, 'float_type');
      | if strcmp(f_type,'custom')
      |     set_param_state(gcb, 'exp_width', 'on')
      |     set_param_state(gcb, 'frac_width', 'on')
      | else
      |     set_param_state(gcb, 'exp_width', 'off')
      |     set_param_state(gcb, 'frac_width', 'off')
      | end
  convert_1_{1..16} (16 alike) : xbsIndex_r4/Convert  gui_display_data_type=Fixed-point  arith_type="Signed  (2's comp)"  n_bits=18  bin_pt=17  float_type=Single  exp_bits=8  fraction_bits=24  quantization="Round  (unbiased: Even Values)"  overflow=Wrap  en=off  latency=1  pipeline=on  dbl_ovrd=off  block_type=convert
  delay1 : xbsIndex_r4/Delay  rst=off  infoeditControl=Selection of Reset will increase slice count due to use of real FFs and instead of SRLs  en=off  latency=1  reg_retiming=off  dbl_ovrd=off  block_type=delay
  edge_detect3 : Subsystem  AncestorBlock=casper_library_misc/edge_detect  mask(edge_detect){edge=Falling, polarity=Active High, x_in=[0 0.08 0.08 0.16 0.16 0.24 0.24 0.32 0.32 0.4], y_in=[-1 -1  1  1  1  1  1  1  1  1], x_out=[0.6 0.68 0.68 0.76 0.76 0.84 0.84 0.92 0.92 1], y_out=[-1 -1  1  1 -1 -1 -1 -1 -1 -1]}
      mask prompts: edge "Edge Type"; polarity "Output Polarity"; x_in "Input X Positions"; y_in "Input Y Positions"; x_out "Output X Positions"; y_out "Output Y Positions"
      mask help: Output is active for one-cycle after each edge of the specified type (i.e. rising, falling or both).
      mask init: same as rfsoc4x2_ospfb_128/edge_detect1
      settings: AttributesFormatString=|
      | falling edges
      | active high
      mask Help: Output is active for one-cycle after each edge of the specified type (i.e. rising, falling, or both).  Latency is zero.
      mask TypeOptions edge: Rising | Falling | Both
      mask TypeOptions polarity: Active High | Active Low
      mask Display:
      | plot(x_in_num,0.5+y_in_num*0.2);
      | plot(x_out_num,0.5+y_out_num*0.2);
  pol1_in10_coeffs : Subsystem  AncestorBlock=casper_library_pfbs/pfb_coeff_gen  mask(pfb_coeff_gen){PFBSize=8, CoeffBitWidth=16, TotalTaps=4, CoeffDistMem=off, WindowType=hamming, bram_latency=2, n_inputs=4, nput=9, fwidth=2, debug_mode=off, fan_latency=1}
      mask prompts: PFBSize "Size of PFB: (2^? pnts)"; CoeffBitWidth "Bitwidth of Coefficients:"; TotalTaps "Total Number of Taps:"; CoeffDistMem "Implement Coeff Gen in Distributed Memory"; WindowType "Windowing Function:"; bram_latency "BRAM Latency"; n_inputs "Number of Simultaneous Inputs: (2^?)"; nput "This is input number:"; fwidth "Bin Width (normal=1)"; debug_mode "Debug mode - coeffs are a [1:pfb_size*taps] ramp."; fan_latency "Fanout latency"
      mask init:
      | pfb_coeff_gen_init(gcb, ...
      |     'PFBSize', PFBSize, ...
      |     'CoeffBitWidth', CoeffBitWidth, ...
      |     'TotalTaps', TotalTaps, ...
      |     'CoeffDistMem', CoeffDistMem, ...
      |     'WindowType', WindowType, ...
      |     'bram_latency', bram_latency, ...
      |     'n_inputs', n_inputs, ...
      |     'nput', nput, ...
      |     'fwidth', fwidth, ...
      |     'fan_latency', fan_latency, ...
      |     'debug_mode', debug_mode);
      settings: AttributesFormatString=|
      | PFBSize=8, n_inputs=4,
      | taps=4, input=9
  pol1_in11_coeffs : Subsystem  AncestorBlock=casper_library_pfbs/pfb_coeff_gen  mask(pfb_coeff_gen){PFBSize=8, CoeffBitWidth=16, TotalTaps=4, CoeffDistMem=off, WindowType=hamming, bram_latency=2, n_inputs=4, nput=10, fwidth=2, debug_mode=off, fan_latency=1}
      mask prompts: PFBSize "Size of PFB: (2^? pnts)"; CoeffBitWidth "Bitwidth of Coefficients:"; TotalTaps "Total Number of Taps:"; CoeffDistMem "Implement Coeff Gen in Distributed Memory"; WindowType "Windowing Function:"; bram_latency "BRAM Latency"; n_inputs "Number of Simultaneous Inputs: (2^?)"; nput "This is input number:"; fwidth "Bin Width (normal=1)"; debug_mode "Debug mode - coeffs are a [1:pfb_size*taps] ramp."; fan_latency "Fanout latency"
      mask init: same as rfsoc4x2_ospfb_128/pfb_fir_real7/pol1_in10_coeffs
      settings: AttributesFormatString=|
      | PFBSize=8, n_inputs=4,
      | taps=4, input=10
  pol1_in12_coeffs : Subsystem  AncestorBlock=casper_library_pfbs/pfb_coeff_gen  mask(pfb_coeff_gen){PFBSize=8, CoeffBitWidth=16, TotalTaps=4, CoeffDistMem=off, WindowType=hamming, bram_latency=2, n_inputs=4, nput=11, fwidth=2, debug_mode=off, fan_latency=1}
      mask prompts: PFBSize "Size of PFB: (2^? pnts)"; CoeffBitWidth "Bitwidth of Coefficients:"; TotalTaps "Total Number of Taps:"; CoeffDistMem "Implement Coeff Gen in Distributed Memory"; WindowType "Windowing Function:"; bram_latency "BRAM Latency"; n_inputs "Number of Simultaneous Inputs: (2^?)"; nput "This is input number:"; fwidth "Bin Width (normal=1)"; debug_mode "Debug mode - coeffs are a [1:pfb_size*taps] ramp."; fan_latency "Fanout latency"
      mask init: same as rfsoc4x2_ospfb_128/pfb_fir_real7/pol1_in10_coeffs
      settings: AttributesFormatString=|
      | PFBSize=8, n_inputs=4,
      | taps=4, input=11
  pol1_in13_coeffs : Subsystem  AncestorBlock=casper_library_pfbs/pfb_coeff_gen  mask(pfb_coeff_gen){PFBSize=8, CoeffBitWidth=16, TotalTaps=4, CoeffDistMem=off, WindowType=hamming, bram_latency=2, n_inputs=4, nput=12, fwidth=2, debug_mode=off, fan_latency=1}
      mask prompts: PFBSize "Size of PFB: (2^? pnts)"; CoeffBitWidth "Bitwidth of Coefficients:"; TotalTaps "Total Number of Taps:"; CoeffDistMem "Implement Coeff Gen in Distributed Memory"; WindowType "Windowing Function:"; bram_latency "BRAM Latency"; n_inputs "Number of Simultaneous Inputs: (2^?)"; nput "This is input number:"; fwidth "Bin Width (normal=1)"; debug_mode "Debug mode - coeffs are a [1:pfb_size*taps] ramp."; fan_latency "Fanout latency"
      mask init: same as rfsoc4x2_ospfb_128/pfb_fir_real7/pol1_in10_coeffs
      settings: AttributesFormatString=|
      | PFBSize=8, n_inputs=4,
      | taps=4, input=12
  pol1_in14_coeffs : Subsystem  AncestorBlock=casper_library_pfbs/pfb_coeff_gen  mask(pfb_coeff_gen){PFBSize=8, CoeffBitWidth=16, TotalTaps=4, CoeffDistMem=off, WindowType=hamming, bram_latency=2, n_inputs=4, nput=13, fwidth=2, debug_mode=off, fan_latency=1}
      mask prompts: PFBSize "Size of PFB: (2^? pnts)"; CoeffBitWidth "Bitwidth of Coefficients:"; TotalTaps "Total Number of Taps:"; CoeffDistMem "Implement Coeff Gen in Distributed Memory"; WindowType "Windowing Function:"; bram_latency "BRAM Latency"; n_inputs "Number of Simultaneous Inputs: (2^?)"; nput "This is input number:"; fwidth "Bin Width (normal=1)"; debug_mode "Debug mode - coeffs are a [1:pfb_size*taps] ramp."; fan_latency "Fanout latency"
      mask init: same as rfsoc4x2_ospfb_128/pfb_fir_real7/pol1_in10_coeffs
      settings: AttributesFormatString=|
      | PFBSize=8, n_inputs=4,
      | taps=4, input=13
  pol1_in15_coeffs : Subsystem  AncestorBlock=casper_library_pfbs/pfb_coeff_gen  mask(pfb_coeff_gen){PFBSize=8, CoeffBitWidth=16, TotalTaps=4, CoeffDistMem=off, WindowType=hamming, bram_latency=2, n_inputs=4, nput=14, fwidth=2, debug_mode=off, fan_latency=1}
      mask prompts: PFBSize "Size of PFB: (2^? pnts)"; CoeffBitWidth "Bitwidth of Coefficients:"; TotalTaps "Total Number of Taps:"; CoeffDistMem "Implement Coeff Gen in Distributed Memory"; WindowType "Windowing Function:"; bram_latency "BRAM Latency"; n_inputs "Number of Simultaneous Inputs: (2^?)"; nput "This is input number:"; fwidth "Bin Width (normal=1)"; debug_mode "Debug mode - coeffs are a [1:pfb_size*taps] ramp."; fan_latency "Fanout latency"
      mask init: same as rfsoc4x2_ospfb_128/pfb_fir_real7/pol1_in10_coeffs
      settings: AttributesFormatString=|
      | PFBSize=8, n_inputs=4,
      | taps=4, input=14
  pol1_in16_coeffs : Subsystem  AncestorBlock=casper_library_pfbs/pfb_coeff_gen  mask(pfb_coeff_gen){PFBSize=8, CoeffBitWidth=16, TotalTaps=4, CoeffDistMem=off, WindowType=hamming, bram_latency=2, n_inputs=4, nput=15, fwidth=2, debug_mode=off, fan_latency=1}
      mask prompts: PFBSize "Size of PFB: (2^? pnts)"; CoeffBitWidth "Bitwidth of Coefficients:"; TotalTaps "Total Number of Taps:"; CoeffDistMem "Implement Coeff Gen in Distributed Memory"; WindowType "Windowing Function:"; bram_latency "BRAM Latency"; n_inputs "Number of Simultaneous Inputs: (2^?)"; nput "This is input number:"; fwidth "Bin Width (normal=1)"; debug_mode "Debug mode - coeffs are a [1:pfb_size*taps] ramp."; fan_latency "Fanout latency"
      mask init: same as rfsoc4x2_ospfb_128/pfb_fir_real7/pol1_in10_coeffs
      settings: AttributesFormatString=|
      | PFBSize=8, n_inputs=4,
      | taps=4, input=15
  pol1_in1_coeffs : Subsystem  AncestorBlock=casper_library_pfbs/pfb_coeff_gen  mask(pfb_coeff_gen){PFBSize=8, CoeffBitWidth=16, TotalTaps=4, CoeffDistMem=off, WindowType=hamming, bram_latency=2, n_inputs=4, nput=0, fwidth=2, debug_mode=off, fan_latency=1}
      mask prompts: PFBSize "Size of PFB: (2^? pnts)"; CoeffBitWidth "Bitwidth of Coefficients:"; TotalTaps "Total Number of Taps:"; CoeffDistMem "Implement Coeff Gen in Distributed Memory"; WindowType "Windowing Function:"; bram_latency "BRAM Latency"; n_inputs "Number of Simultaneous Inputs: (2^?)"; nput "This is input number:"; fwidth "Bin Width (normal=1)"; debug_mode "Debug mode - coeffs are a [1:pfb_size*taps] ramp."; fan_latency "Fanout latency"
      mask init: same as rfsoc4x2_ospfb_128/pfb_fir_real7/pol1_in10_coeffs
      settings: AttributesFormatString=|
      | PFBSize=8, n_inputs=4,
      | taps=4, input=0
  pol1_in1_first_tap : Subsystem  AncestorBlock=casper_library_pfbs/first_tap_real  mask(first_tap_real){PFBSize=8, n_pol_blocks=1, CoeffBitWidth=16, TotalTaps=4, BitWidthIn=16, WindowType=hamming, mult_latency=2, bram_latency=2, n_inputs=4, fwidth=2, use_hdl=on, use_embedded=off}
      mask prompts: PFBSize "Size of PFB: (2^? pnts)"; n_pol_blocks "Number of serial polarization blocks"; CoeffBitWidth "Bitwidth of Coefficients:"; TotalTaps "Total Number of Taps:"; BitWidthIn "Input Bitwidth:"; WindowType "Windowing Function:"; mult_latency "Mult Latency"; bram_latency "BRAM Latency"; n_inputs "Number of Simultaneous Inputs: (2^?)"; fwidth "Bit Width (normal=1)"; use_hdl "Use behavioral HDL for multlipliers"; use_embedded "Use embedded multipliers"
      mask init:
      | first_tap_real_init(gcb,...
      |     'PFBSize', PFBSize,...
      |     'CoeffBitWidth', CoeffBitWidth,...
      |     'TotalTaps', TotalTaps,...
      |     'BitWidthIn', BitWidthIn,...
      |     'WindowType', WindowType,...
      |     'mult_latency', mult_latency,...
      |     'bram_latency', bram_latency,...
      |     'n_inputs', n_inputs,...
      |     'n_pol_blocks', n_pol_blocks, ...
      |     'fwidth', fwidth,...
      |     'use_hdl', use_hdl,...
      |     'use_embedded', use_embedded);
      settings: AttributesFormatString=taps=4
      mask TypeOptions WindowType: bartlett | barthannwin | blackman | blackmanharris | bohamwin | chebwin | flattopwin | gausswin | hamming | hann | kaiser | nuttallwin | parzenwin | rectwin | tukeywin | triang | userwindow
      mask Callback use_hdl:
      | use_hdl = get_param(gcb,'use_hdl');
      | if( strcmp(use_hdl,'on')),
      |     set_param(gcb, 'use_embedded','off');
      |     set_param(gcb, 'MaskVisibilities',{'on','on','on','on','on','on','on','on','on','on','on','off'});
      | else,
      |     set_param(gcb, 'MaskVisibilities',{'on','on','on','on','on','on','on','on','on','on','on','on'});
      | end
  pol1_in1_first_tap1 : Subsystem  AncestorBlock=casper_library_pfbs/first_tap_real  mask(first_tap_real){PFBSize=8, n_pol_blocks=1, CoeffBitWidth=16, TotalTaps=4, BitWidthIn=16, WindowType=hamming, mult_latency=2, bram_latency=2, n_inputs=4, fwidth=2, use_hdl=on, use_embedded=off}
      mask prompts: PFBSize "Size of PFB: (2^? pnts)"; n_pol_blocks "Number of serial polarization blocks"; CoeffBitWidth "Bitwidth of Coefficients:"; TotalTaps "Total Number of Taps:"; BitWidthIn "Input Bitwidth:"; WindowType "Windowing Function:"; mult_latency "Mult Latency"; bram_latency "BRAM Latency"; n_inputs "Number of Simultaneous Inputs: (2^?)"; fwidth "Bit Width (normal=1)"; use_hdl "Use behavioral HDL for multlipliers"; use_embedded "Use embedded multipliers"
      mask init: same as rfsoc4x2_ospfb_128/pfb_fir_real7/pol1_in1_first_tap
      settings: AttributesFormatString=taps=4
      mask TypeOptions WindowType: bartlett | barthannwin | blackman | blackmanharris | bohamwin | chebwin | flattopwin | gausswin | hamming | hann | kaiser | nuttallwin | parzenwin | rectwin | tukeywin | triang | userwindow
      mask Callback use_hdl:
      | use_hdl = get_param(gcb,'use_hdl');
      | if( strcmp(use_hdl,'on')),
      |     set_param(gcb, 'use_embedded','off');
      |     set_param(gcb, 'MaskVisibilities',{'on','on','on','on','on','on','on','on','on','on','on','off'});
      | else,
      |     set_param(gcb, 'MaskVisibilities',{'on','on','on','on','on','on','on','on','on','on','on','on'});
      | end
  pol1_in1_first_tap10 : Subsystem  AncestorBlock=casper_library_pfbs/first_tap_real  mask(first_tap_real){PFBSize=8, n_pol_blocks=1, CoeffBitWidth=16, TotalTaps=4, BitWidthIn=16, WindowType=hamming, mult_latency=2, bram_latency=2, n_inputs=4, fwidth=2, use_hdl=on, use_embedded=off}
      mask prompts: PFBSize "Size of PFB: (2^? pnts)"; n_pol_blocks "Number of serial polarization blocks"; CoeffBitWidth "Bitwidth of Coefficients:"; TotalTaps "Total Number of Taps:"; BitWidthIn "Input Bitwidth:"; WindowType "Windowing Function:"; mult_latency "Mult Latency"; bram_latency "BRAM Latency"; n_inputs "Number of Simultaneous Inputs: (2^?)"; fwidth "Bit Width (normal=1)"; use_hdl "Use behavioral HDL for multlipliers"; use_embedded "Use embedded multipliers"
      mask init: same as rfsoc4x2_ospfb_128/pfb_fir_real7/pol1_in1_first_tap
      settings: AttributesFormatString=taps=4
      mask TypeOptions WindowType: bartlett | barthannwin | blackman | blackmanharris | bohamwin | chebwin | flattopwin | gausswin | hamming | hann | kaiser | nuttallwin | parzenwin | rectwin | tukeywin | triang | userwindow
      mask Callback use_hdl:
      | use_hdl = get_param(gcb,'use_hdl');
      | if( strcmp(use_hdl,'on')),
      |     set_param(gcb, 'use_embedded','off');
      |     set_param(gcb, 'MaskVisibilities',{'on','on','on','on','on','on','on','on','on','on','on','off'});
      | else,
      |     set_param(gcb, 'MaskVisibilities',{'on','on','on','on','on','on','on','on','on','on','on','on'});
      | end
  pol1_in1_first_tap11 : Subsystem  AncestorBlock=casper_library_pfbs/first_tap_real  mask(first_tap_real){PFBSize=8, n_pol_blocks=1, CoeffBitWidth=16, TotalTaps=4, BitWidthIn=16, WindowType=hamming, mult_latency=2, bram_latency=2, n_inputs=4, fwidth=2, use_hdl=on, use_embedded=off}
      mask prompts: PFBSize "Size of PFB: (2^? pnts)"; n_pol_blocks "Number of serial polarization blocks"; CoeffBitWidth "Bitwidth of Coefficients:"; TotalTaps "Total Number of Taps:"; BitWidthIn "Input Bitwidth:"; WindowType "Windowing Function:"; mult_latency "Mult Latency"; bram_latency "BRAM Latency"; n_inputs "Number of Simultaneous Inputs: (2^?)"; fwidth "Bit Width (normal=1)"; use_hdl "Use behavioral HDL for multlipliers"; use_embedded "Use embedded multipliers"
      mask init: same as rfsoc4x2_ospfb_128/pfb_fir_real7/pol1_in1_first_tap
      settings: AttributesFormatString=taps=4
      mask TypeOptions WindowType: bartlett | barthannwin | blackman | blackmanharris | bohamwin | chebwin | flattopwin | gausswin | hamming | hann | kaiser | nuttallwin | parzenwin | rectwin | tukeywin | triang | userwindow
      mask Callback use_hdl:
      | use_hdl = get_param(gcb,'use_hdl');
      | if( strcmp(use_hdl,'on')),
      |     set_param(gcb, 'use_embedded','off');
      |     set_param(gcb, 'MaskVisibilities',{'on','on','on','on','on','on','on','on','on','on','on','off'});
      | else,
      |     set_param(gcb, 'MaskVisibilities',{'on','on','on','on','on','on','on','on','on','on','on','on'});
      | end
  pol1_in1_first_tap12 : Subsystem  AncestorBlock=casper_library_pfbs/first_tap_real  mask(first_tap_real){PFBSize=8, n_pol_blocks=1, CoeffBitWidth=16, TotalTaps=4, BitWidthIn=16, WindowType=hamming, mult_latency=2, bram_latency=2, n_inputs=4, fwidth=2, use_hdl=on, use_embedded=off}
      mask prompts: PFBSize "Size of PFB: (2^? pnts)"; n_pol_blocks "Number of serial polarization blocks"; CoeffBitWidth "Bitwidth of Coefficients:"; TotalTaps "Total Number of Taps:"; BitWidthIn "Input Bitwidth:"; WindowType "Windowing Function:"; mult_latency "Mult Latency"; bram_latency "BRAM Latency"; n_inputs "Number of Simultaneous Inputs: (2^?)"; fwidth "Bit Width (normal=1)"; use_hdl "Use behavioral HDL for multlipliers"; use_embedded "Use embedded multipliers"
      mask init: same as rfsoc4x2_ospfb_128/pfb_fir_real7/pol1_in1_first_tap
      settings: AttributesFormatString=taps=4
      mask TypeOptions WindowType: bartlett | barthannwin | blackman | blackmanharris | bohamwin | chebwin | flattopwin | gausswin | hamming | hann | kaiser | nuttallwin | parzenwin | rectwin | tukeywin | triang | userwindow
      mask Callback use_hdl:
      | use_hdl = get_param(gcb,'use_hdl');
      | if( strcmp(use_hdl,'on')),
      |     set_param(gcb, 'use_embedded','off');
      |     set_param(gcb, 'MaskVisibilities',{'on','on','on','on','on','on','on','on','on','on','on','off'});
      | else,
      |     set_param(gcb, 'MaskVisibilities',{'on','on','on','on','on','on','on','on','on','on','on','on'});
      | end
  pol1_in1_first_tap13 : Subsystem  AncestorBlock=casper_library_pfbs/first_tap_real  mask(first_tap_real){PFBSize=8, n_pol_blocks=1, CoeffBitWidth=16, TotalTaps=4, BitWidthIn=16, WindowType=hamming, mult_latency=2, bram_latency=2, n_inputs=4, fwidth=2, use_hdl=on, use_embedded=off}
      mask prompts: PFBSize "Size of PFB: (2^? pnts)"; n_pol_blocks "Number of serial polarization blocks"; CoeffBitWidth "Bitwidth of Coefficients:"; TotalTaps "Total Number of Taps:"; BitWidthIn "Input Bitwidth:"; WindowType "Windowing Function:"; mult_latency "Mult Latency"; bram_latency "BRAM Latency"; n_inputs "Number of Simultaneous Inputs: (2^?)"; fwidth "Bit Width (normal=1)"; use_hdl "Use behavioral HDL for multlipliers"; use_embedded "Use embedded multipliers"
      mask init: same as rfsoc4x2_ospfb_128/pfb_fir_real7/pol1_in1_first_tap
      settings: AttributesFormatString=taps=4
      mask TypeOptions WindowType: bartlett | barthannwin | blackman | blackmanharris | bohamwin | chebwin | flattopwin | gausswin | hamming | hann | kaiser | nuttallwin | parzenwin | rectwin | tukeywin | triang | userwindow
      mask Callback use_hdl:
      | use_hdl = get_param(gcb,'use_hdl');
      | if( strcmp(use_hdl,'on')),
      |     set_param(gcb, 'use_embedded','off');
      |     set_param(gcb, 'MaskVisibilities',{'on','on','on','on','on','on','on','on','on','on','on','off'});
      | else,
      |     set_param(gcb, 'MaskVisibilities',{'on','on','on','on','on','on','on','on','on','on','on','on'});
      | end
  pol1_in1_first_tap14 : Subsystem  AncestorBlock=casper_library_pfbs/first_tap_real  mask(first_tap_real){PFBSize=8, n_pol_blocks=1, CoeffBitWidth=16, TotalTaps=4, BitWidthIn=16, WindowType=hamming, mult_latency=2, bram_latency=2, n_inputs=4, fwidth=2, use_hdl=on, use_embedded=off}
      mask prompts: PFBSize "Size of PFB: (2^? pnts)"; n_pol_blocks "Number of serial polarization blocks"; CoeffBitWidth "Bitwidth of Coefficients:"; TotalTaps "Total Number of Taps:"; BitWidthIn "Input Bitwidth:"; WindowType "Windowing Function:"; mult_latency "Mult Latency"; bram_latency "BRAM Latency"; n_inputs "Number of Simultaneous Inputs: (2^?)"; fwidth "Bit Width (normal=1)"; use_hdl "Use behavioral HDL for multlipliers"; use_embedded "Use embedded multipliers"
      mask init: same as rfsoc4x2_ospfb_128/pfb_fir_real7/pol1_in1_first_tap
      settings: AttributesFormatString=taps=4
      mask TypeOptions WindowType: bartlett | barthannwin | blackman | blackmanharris | bohamwin | chebwin | flattopwin | gausswin | hamming | hann | kaiser | nuttallwin | parzenwin | rectwin | tukeywin | triang | userwindow
      mask Callback use_hdl:
      | use_hdl = get_param(gcb,'use_hdl');
      | if( strcmp(use_hdl,'on')),
      |     set_param(gcb, 'use_embedded','off');
      |     set_param(gcb, 'MaskVisibilities',{'on','on','on','on','on','on','on','on','on','on','on','off'});
      | else,
      |     set_param(gcb, 'MaskVisibilities',{'on','on','on','on','on','on','on','on','on','on','on','on'});
      | end
  pol1_in1_first_tap15 : Subsystem  AncestorBlock=casper_library_pfbs/first_tap_real  mask(first_tap_real){PFBSize=8, n_pol_blocks=1, CoeffBitWidth=16, TotalTaps=4, BitWidthIn=16, WindowType=hamming, mult_latency=2, bram_latency=2, n_inputs=4, fwidth=2, use_hdl=on, use_embedded=off}
      mask prompts: PFBSize "Size of PFB: (2^? pnts)"; n_pol_blocks "Number of serial polarization blocks"; CoeffBitWidth "Bitwidth of Coefficients:"; TotalTaps "Total Number of Taps:"; BitWidthIn "Input Bitwidth:"; WindowType "Windowing Function:"; mult_latency "Mult Latency"; bram_latency "BRAM Latency"; n_inputs "Number of Simultaneous Inputs: (2^?)"; fwidth "Bit Width (normal=1)"; use_hdl "Use behavioral HDL for multlipliers"; use_embedded "Use embedded multipliers"
      mask init: same as rfsoc4x2_ospfb_128/pfb_fir_real7/pol1_in1_first_tap
      settings: AttributesFormatString=taps=4
      mask TypeOptions WindowType: bartlett | barthannwin | blackman | blackmanharris | bohamwin | chebwin | flattopwin | gausswin | hamming | hann | kaiser | nuttallwin | parzenwin | rectwin | tukeywin | triang | userwindow
      mask Callback use_hdl:
      | use_hdl = get_param(gcb,'use_hdl');
      | if( strcmp(use_hdl,'on')),
      |     set_param(gcb, 'use_embedded','off');
      |     set_param(gcb, 'MaskVisibilities',{'on','on','on','on','on','on','on','on','on','on','on','off'});
      | else,
      |     set_param(gcb, 'MaskVisibilities',{'on','on','on','on','on','on','on','on','on','on','on','on'});
      | end
  pol1_in1_first_tap2 : Subsystem  AncestorBlock=casper_library_pfbs/first_tap_real  mask(first_tap_real){PFBSize=8, n_pol_blocks=1, CoeffBitWidth=16, TotalTaps=4, BitWidthIn=16, WindowType=hamming, mult_latency=2, bram_latency=2, n_inputs=4, fwidth=2, use_hdl=on, use_embedded=off}
      mask prompts: PFBSize "Size of PFB: (2^? pnts)"; n_pol_blocks "Number of serial polarization blocks"; CoeffBitWidth "Bitwidth of Coefficients:"; TotalTaps "Total Number of Taps:"; BitWidthIn "Input Bitwidth:"; WindowType "Windowing Function:"; mult_latency "Mult Latency"; bram_latency "BRAM Latency"; n_inputs "Number of Simultaneous Inputs: (2^?)"; fwidth "Bit Width (normal=1)"; use_hdl "Use behavioral HDL for multlipliers"; use_embedded "Use embedded multipliers"
      mask init: same as rfsoc4x2_ospfb_128/pfb_fir_real7/pol1_in1_first_tap
      settings: AttributesFormatString=taps=4
      mask TypeOptions WindowType: bartlett | barthannwin | blackman | blackmanharris | bohamwin | chebwin | flattopwin | gausswin | hamming | hann | kaiser | nuttallwin | parzenwin | rectwin | tukeywin | triang | userwindow
      mask Callback use_hdl:
      | use_hdl = get_param(gcb,'use_hdl');
      | if( strcmp(use_hdl,'on')),
      |     set_param(gcb, 'use_embedded','off');
      |     set_param(gcb, 'MaskVisibilities',{'on','on','on','on','on','on','on','on','on','on','on','off'});
      | else,
      |     set_param(gcb, 'MaskVisibilities',{'on','on','on','on','on','on','on','on','on','on','on','on'});
      | end
  pol1_in1_first_tap3 : Subsystem  AncestorBlock=casper_library_pfbs/first_tap_real  mask(first_tap_real){PFBSize=8, n_pol_blocks=1, CoeffBitWidth=16, TotalTaps=4, BitWidthIn=16, WindowType=hamming, mult_latency=2, bram_latency=2, n_inputs=4, fwidth=2, use_hdl=on, use_embedded=off}
      mask prompts: PFBSize "Size of PFB: (2^? pnts)"; n_pol_blocks "Number of serial polarization blocks"; CoeffBitWidth "Bitwidth of Coefficients:"; TotalTaps "Total Number of Taps:"; BitWidthIn "Input Bitwidth:"; WindowType "Windowing Function:"; mult_latency "Mult Latency"; bram_latency "BRAM Latency"; n_inputs "Number of Simultaneous Inputs: (2^?)"; fwidth "Bit Width (normal=1)"; use_hdl "Use behavioral HDL for multlipliers"; use_embedded "Use embedded multipliers"
      mask init: same as rfsoc4x2_ospfb_128/pfb_fir_real7/pol1_in1_first_tap
      settings: AttributesFormatString=taps=4
      mask TypeOptions WindowType: bartlett | barthannwin | blackman | blackmanharris | bohamwin | chebwin | flattopwin | gausswin | hamming | hann | kaiser | nuttallwin | parzenwin | rectwin | tukeywin | triang | userwindow
      mask Callback use_hdl:
      | use_hdl = get_param(gcb,'use_hdl');
      | if( strcmp(use_hdl,'on')),
      |     set_param(gcb, 'use_embedded','off');
      |     set_param(gcb, 'MaskVisibilities',{'on','on','on','on','on','on','on','on','on','on','on','off'});
      | else,
      |     set_param(gcb, 'MaskVisibilities',{'on','on','on','on','on','on','on','on','on','on','on','on'});
      | end
  pol1_in1_first_tap4 : Subsystem  AncestorBlock=casper_library_pfbs/first_tap_real  mask(first_tap_real){PFBSize=8, n_pol_blocks=1, CoeffBitWidth=16, TotalTaps=4, BitWidthIn=16, WindowType=hamming, mult_latency=2, bram_latency=2, n_inputs=4, fwidth=2, use_hdl=on, use_embedded=off}
      mask prompts: PFBSize "Size of PFB: (2^? pnts)"; n_pol_blocks "Number of serial polarization blocks"; CoeffBitWidth "Bitwidth of Coefficients:"; TotalTaps "Total Number of Taps:"; BitWidthIn "Input Bitwidth:"; WindowType "Windowing Function:"; mult_latency "Mult Latency"; bram_latency "BRAM Latency"; n_inputs "Number of Simultaneous Inputs: (2^?)"; fwidth "Bit Width (normal=1)"; use_hdl "Use behavioral HDL for multlipliers"; use_embedded "Use embedded multipliers"
      mask init: same as rfsoc4x2_ospfb_128/pfb_fir_real7/pol1_in1_first_tap
      settings: AttributesFormatString=taps=4
      mask TypeOptions WindowType: bartlett | barthannwin | blackman | blackmanharris | bohamwin | chebwin | flattopwin | gausswin | hamming | hann | kaiser | nuttallwin | parzenwin | rectwin | tukeywin | triang | userwindow
      mask Callback use_hdl:
      | use_hdl = get_param(gcb,'use_hdl');
      | if( strcmp(use_hdl,'on')),
      |     set_param(gcb, 'use_embedded','off');
      |     set_param(gcb, 'MaskVisibilities',{'on','on','on','on','on','on','on','on','on','on','on','off'});
      | else,
      |     set_param(gcb, 'MaskVisibilities',{'on','on','on','on','on','on','on','on','on','on','on','on'});
      | end
  pol1_in1_first_tap5 : Subsystem  AncestorBlock=casper_library_pfbs/first_tap_real  mask(first_tap_real){PFBSize=8, n_pol_blocks=1, CoeffBitWidth=16, TotalTaps=4, BitWidthIn=16, WindowType=hamming, mult_latency=2, bram_latency=2, n_inputs=4, fwidth=2, use_hdl=on, use_embedded=off}
      mask prompts: PFBSize "Size of PFB: (2^? pnts)"; n_pol_blocks "Number of serial polarization blocks"; CoeffBitWidth "Bitwidth of Coefficients:"; TotalTaps "Total Number of Taps:"; BitWidthIn "Input Bitwidth:"; WindowType "Windowing Function:"; mult_latency "Mult Latency"; bram_latency "BRAM Latency"; n_inputs "Number of Simultaneous Inputs: (2^?)"; fwidth "Bit Width (normal=1)"; use_hdl "Use behavioral HDL for multlipliers"; use_embedded "Use embedded multipliers"
      mask init: same as rfsoc4x2_ospfb_128/pfb_fir_real7/pol1_in1_first_tap
      settings: AttributesFormatString=taps=4
      mask TypeOptions WindowType: bartlett | barthannwin | blackman | blackmanharris | bohamwin | chebwin | flattopwin | gausswin | hamming | hann | kaiser | nuttallwin | parzenwin | rectwin | tukeywin | triang | userwindow
      mask Callback use_hdl:
      | use_hdl = get_param(gcb,'use_hdl');
      | if( strcmp(use_hdl,'on')),
      |     set_param(gcb, 'use_embedded','off');
      |     set_param(gcb, 'MaskVisibilities',{'on','on','on','on','on','on','on','on','on','on','on','off'});
      | else,
      |     set_param(gcb, 'MaskVisibilities',{'on','on','on','on','on','on','on','on','on','on','on','on'});
      | end
  pol1_in1_first_tap6 : Subsystem  AncestorBlock=casper_library_pfbs/first_tap_real  mask(first_tap_real){PFBSize=8, n_pol_blocks=1, CoeffBitWidth=16, TotalTaps=4, BitWidthIn=16, WindowType=hamming, mult_latency=2, bram_latency=2, n_inputs=4, fwidth=2, use_hdl=on, use_embedded=off}
      mask prompts: PFBSize "Size of PFB: (2^? pnts)"; n_pol_blocks "Number of serial polarization blocks"; CoeffBitWidth "Bitwidth of Coefficients:"; TotalTaps "Total Number of Taps:"; BitWidthIn "Input Bitwidth:"; WindowType "Windowing Function:"; mult_latency "Mult Latency"; bram_latency "BRAM Latency"; n_inputs "Number of Simultaneous Inputs: (2^?)"; fwidth "Bit Width (normal=1)"; use_hdl "Use behavioral HDL for multlipliers"; use_embedded "Use embedded multipliers"
      mask init: same as rfsoc4x2_ospfb_128/pfb_fir_real7/pol1_in1_first_tap
      settings: AttributesFormatString=taps=4
      mask TypeOptions WindowType: bartlett | barthannwin | blackman | blackmanharris | bohamwin | chebwin | flattopwin | gausswin | hamming | hann | kaiser | nuttallwin | parzenwin | rectwin | tukeywin | triang | userwindow
      mask Callback use_hdl:
      | use_hdl = get_param(gcb,'use_hdl');
      | if( strcmp(use_hdl,'on')),
      |     set_param(gcb, 'use_embedded','off');
      |     set_param(gcb, 'MaskVisibilities',{'on','on','on','on','on','on','on','on','on','on','on','off'});
      | else,
      |     set_param(gcb, 'MaskVisibilities',{'on','on','on','on','on','on','on','on','on','on','on','on'});
      | end
  pol1_in1_first_tap7 : Subsystem  AncestorBlock=casper_library_pfbs/first_tap_real  mask(first_tap_real){PFBSize=8, n_pol_blocks=1, CoeffBitWidth=16, TotalTaps=4, BitWidthIn=16, WindowType=hamming, mult_latency=2, bram_latency=2, n_inputs=4, fwidth=2, use_hdl=on, use_embedded=off}
      mask prompts: PFBSize "Size of PFB: (2^? pnts)"; n_pol_blocks "Number of serial polarization blocks"; CoeffBitWidth "Bitwidth of Coefficients:"; TotalTaps "Total Number of Taps:"; BitWidthIn "Input Bitwidth:"; WindowType "Windowing Function:"; mult_latency "Mult Latency"; bram_latency "BRAM Latency"; n_inputs "Number of Simultaneous Inputs: (2^?)"; fwidth "Bit Width (normal=1)"; use_hdl "Use behavioral HDL for multlipliers"; use_embedded "Use embedded multipliers"
      mask init: same as rfsoc4x2_ospfb_128/pfb_fir_real7/pol1_in1_first_tap
      settings: AttributesFormatString=taps=4
      mask TypeOptions WindowType: bartlett | barthannwin | blackman | blackmanharris | bohamwin | chebwin | flattopwin | gausswin | hamming | hann | kaiser | nuttallwin | parzenwin | rectwin | tukeywin | triang | userwindow
      mask Callback use_hdl:
      | use_hdl = get_param(gcb,'use_hdl');
      | if( strcmp(use_hdl,'on')),
      |     set_param(gcb, 'use_embedded','off');
      |     set_param(gcb, 'MaskVisibilities',{'on','on','on','on','on','on','on','on','on','on','on','off'});
      | else,
      |     set_param(gcb, 'MaskVisibilities',{'on','on','on','on','on','on','on','on','on','on','on','on'});
      | end
  pol1_in1_first_tap8 : Subsystem  AncestorBlock=casper_library_pfbs/first_tap_real  mask(first_tap_real){PFBSize=8, n_pol_blocks=1, CoeffBitWidth=16, TotalTaps=4, BitWidthIn=16, WindowType=hamming, mult_latency=2, bram_latency=2, n_inputs=4, fwidth=2, use_hdl=on, use_embedded=off}
      mask prompts: PFBSize "Size of PFB: (2^? pnts)"; n_pol_blocks "Number of serial polarization blocks"; CoeffBitWidth "Bitwidth of Coefficients:"; TotalTaps "Total Number of Taps:"; BitWidthIn "Input Bitwidth:"; WindowType "Windowing Function:"; mult_latency "Mult Latency"; bram_latency "BRAM Latency"; n_inputs "Number of Simultaneous Inputs: (2^?)"; fwidth "Bit Width (normal=1)"; use_hdl "Use behavioral HDL for multlipliers"; use_embedded "Use embedded multipliers"
      mask init: same as rfsoc4x2_ospfb_128/pfb_fir_real7/pol1_in1_first_tap
      settings: AttributesFormatString=taps=4
      mask TypeOptions WindowType: bartlett | barthannwin | blackman | blackmanharris | bohamwin | chebwin | flattopwin | gausswin | hamming | hann | kaiser | nuttallwin | parzenwin | rectwin | tukeywin | triang | userwindow
      mask Callback use_hdl:
      | use_hdl = get_param(gcb,'use_hdl');
      | if( strcmp(use_hdl,'on')),
      |     set_param(gcb, 'use_embedded','off');
      |     set_param(gcb, 'MaskVisibilities',{'on','on','on','on','on','on','on','on','on','on','on','off'});
      | else,
      |     set_param(gcb, 'MaskVisibilities',{'on','on','on','on','on','on','on','on','on','on','on','on'});
      | end
  pol1_in1_first_tap9 : Subsystem  AncestorBlock=casper_library_pfbs/first_tap_real  mask(first_tap_real){PFBSize=8, n_pol_blocks=1, CoeffBitWidth=16, TotalTaps=4, BitWidthIn=16, WindowType=hamming, mult_latency=2, bram_latency=2, n_inputs=4, fwidth=2, use_hdl=on, use_embedded=off}
      mask prompts: PFBSize "Size of PFB: (2^? pnts)"; n_pol_blocks "Number of serial polarization blocks"; CoeffBitWidth "Bitwidth of Coefficients:"; TotalTaps "Total Number of Taps:"; BitWidthIn "Input Bitwidth:"; WindowType "Windowing Function:"; mult_latency "Mult Latency"; bram_latency "BRAM Latency"; n_inputs "Number of Simultaneous Inputs: (2^?)"; fwidth "Bit Width (normal=1)"; use_hdl "Use behavioral HDL for multlipliers"; use_embedded "Use embedded multipliers"
      mask init: same as rfsoc4x2_ospfb_128/pfb_fir_real7/pol1_in1_first_tap
      settings: AttributesFormatString=taps=4
      mask TypeOptions WindowType: bartlett | barthannwin | blackman | blackmanharris | bohamwin | chebwin | flattopwin | gausswin | hamming | hann | kaiser | nuttallwin | parzenwin | rectwin | tukeywin | triang | userwindow
      mask Callback use_hdl:
      | use_hdl = get_param(gcb,'use_hdl');
      | if( strcmp(use_hdl,'on')),
      |     set_param(gcb, 'use_embedded','off');
      |     set_param(gcb, 'MaskVisibilities',{'on','on','on','on','on','on','on','on','on','on','on','off'});
      | else,
      |     set_param(gcb, 'MaskVisibilities',{'on','on','on','on','on','on','on','on','on','on','on','on'});
      | end
  pol1_in1_last_tap : Subsystem  AncestorBlock=casper_library_pfbs/last_tap_real  mask(last_tap_real){BitWidthIn=16, CoeffBitWidth=16, mult_latency=2, use_hdl=on, use_embedded=off}
      mask prompts: BitWidthIn "Input Bitwidth:"; CoeffBitWidth "Coeff Bitwidth:"; mult_latency "Mult Latency"; use_hdl "Use behavioral HDL for multlipliers"; use_embedded "Use embedded multipliers"
      mask init:
      | last_tap_real_init(gcb,...
      |     'BitWidthIn', BitWidthIn,...
      |     'CoeffBitWidth', CoeffBitWidth,...
      |     'mult_latency', mult_latency,...
      |     'use_hdl', use_hdl,...
      |     'use_embedded', use_embedded);
      mask Callback use_hdl:
      | use_hdl = get_param(gcb,'use_hdl');
      | if( strcmp(use_hdl,'on')),
      |     set_param(gcb, 'use_embedded','off');
      |     set_param(gcb, 'MaskVisibilities',{'on','on','on','on','off'});
      | else,
      |     set_param(gcb, 'MaskVisibilities',{'on','on','on','on','on'});
      | end
  pol1_in1_last_tap1 : Subsystem  AncestorBlock=casper_library_pfbs/last_tap_real  mask(last_tap_real){BitWidthIn=16, CoeffBitWidth=16, mult_latency=2, use_hdl=on, use_embedded=off}
      mask prompts: BitWidthIn "Input Bitwidth:"; CoeffBitWidth "Coeff Bitwidth:"; mult_latency "Mult Latency"; use_hdl "Use behavioral HDL for multlipliers"; use_embedded "Use embedded multipliers"
      mask init:
      | last_tap_real_init(gcb,...
      |     'BitWidthIn', BitWidthIn,...
      |     'CoeffBitWidth', CoeffBitWidth,...
      |     'mult_latency', mult_latency,...
      |     'use_hdl', use_hdl,...
      |     'use_embedded', use_embedded);
      mask Callback use_hdl:
      | use_hdl = get_param(gcb,'use_hdl');
      | if( strcmp(use_hdl,'on')),
      |     set_param(gcb, 'use_embedded','off');
      |     set_param(gcb, 'MaskVisibilities',{'on','on','on','on','off'});
      | else,
      |     set_param(gcb, 'MaskVisibilities',{'on','on','on','on','on'});
      | end
  pol1_in1_last_tap10 : Subsystem  AncestorBlock=casper_library_pfbs/last_tap_real  mask(last_tap_real){BitWidthIn=16, CoeffBitWidth=16, mult_latency=2, use_hdl=on, use_embedded=off}
      mask prompts: BitWidthIn "Input Bitwidth:"; CoeffBitWidth "Coeff Bitwidth:"; mult_latency "Mult Latency"; use_hdl "Use behavioral HDL for multlipliers"; use_embedded "Use embedded multipliers"
      mask init:
      | last_tap_real_init(gcb,...
      |     'BitWidthIn', BitWidthIn,...
      |     'CoeffBitWidth', CoeffBitWidth,...
      |     'mult_latency', mult_latency,...
      |     'use_hdl', use_hdl,...
      |     'use_embedded', use_embedded);
      mask Callback use_hdl:
      | use_hdl = get_param(gcb,'use_hdl');
      | if( strcmp(use_hdl,'on')),
      |     set_param(gcb, 'use_embedded','off');
      |     set_param(gcb, 'MaskVisibilities',{'on','on','on','on','off'});
      | else,
      |     set_param(gcb, 'MaskVisibilities',{'on','on','on','on','on'});
      | end
  pol1_in1_last_tap11 : Subsystem  AncestorBlock=casper_library_pfbs/last_tap_real  mask(last_tap_real){BitWidthIn=16, CoeffBitWidth=16, mult_latency=2, use_hdl=on, use_embedded=off}
      mask prompts: BitWidthIn "Input Bitwidth:"; CoeffBitWidth "Coeff Bitwidth:"; mult_latency "Mult Latency"; use_hdl "Use behavioral HDL for multlipliers"; use_embedded "Use embedded multipliers"
      mask init:
      | last_tap_real_init(gcb,...
      |     'BitWidthIn', BitWidthIn,...
      |     'CoeffBitWidth', CoeffBitWidth,...
      |     'mult_latency', mult_latency,...
      |     'use_hdl', use_hdl,...
      |     'use_embedded', use_embedded);
      mask Callback use_hdl:
      | use_hdl = get_param(gcb,'use_hdl');
      | if( strcmp(use_hdl,'on')),
      |     set_param(gcb, 'use_embedded','off');
      |     set_param(gcb, 'MaskVisibilities',{'on','on','on','on','off'});
      | else,
      |     set_param(gcb, 'MaskVisibilities',{'on','on','on','on','on'});
      | end
  pol1_in1_last_tap12 : Subsystem  AncestorBlock=casper_library_pfbs/last_tap_real  mask(last_tap_real){BitWidthIn=16, CoeffBitWidth=16, mult_latency=2, use_hdl=on, use_embedded=off}
      mask prompts: BitWidthIn "Input Bitwidth:"; CoeffBitWidth "Coeff Bitwidth:"; mult_latency "Mult Latency"; use_hdl "Use behavioral HDL for multlipliers"; use_embedded "Use embedded multipliers"
      mask init:
      | last_tap_real_init(gcb,...
      |     'BitWidthIn', BitWidthIn,...
      |     'CoeffBitWidth', CoeffBitWidth,...
      |     'mult_latency', mult_latency,...
      |     'use_hdl', use_hdl,...
      |     'use_embedded', use_embedded);
      mask Callback use_hdl:
      | use_hdl = get_param(gcb,'use_hdl');
      | if( strcmp(use_hdl,'on')),
      |     set_param(gcb, 'use_embedded','off');
      |     set_param(gcb, 'MaskVisibilities',{'on','on','on','on','off'});
      | else,
      |     set_param(gcb, 'MaskVisibilities',{'on','on','on','on','on'});
      | end
  pol1_in1_last_tap13 : Subsystem  AncestorBlock=casper_library_pfbs/last_tap_real  mask(last_tap_real){BitWidthIn=16, CoeffBitWidth=16, mult_latency=2, use_hdl=on, use_embedded=off}
      mask prompts: BitWidthIn "Input Bitwidth:"; CoeffBitWidth "Coeff Bitwidth:"; mult_latency "Mult Latency"; use_hdl "Use behavioral HDL for multlipliers"; use_embedded "Use embedded multipliers"
      mask init:
      | last_tap_real_init(gcb,...
      |     'BitWidthIn', BitWidthIn,...
      |     'CoeffBitWidth', CoeffBitWidth,...
      |     'mult_latency', mult_latency,...
      |     'use_hdl', use_hdl,...
      |     'use_embedded', use_embedded);
      mask Callback use_hdl:
      | use_hdl = get_param(gcb,'use_hdl');
      | if( strcmp(use_hdl,'on')),
      |     set_param(gcb, 'use_embedded','off');
      |     set_param(gcb, 'MaskVisibilities',{'on','on','on','on','off'});
      | else,
      |     set_param(gcb, 'MaskVisibilities',{'on','on','on','on','on'});
      | end
  pol1_in1_last_tap14 : Subsystem  AncestorBlock=casper_library_pfbs/last_tap_real  mask(last_tap_real){BitWidthIn=16, CoeffBitWidth=16, mult_latency=2, use_hdl=on, use_embedded=off}
      mask prompts: BitWidthIn "Input Bitwidth:"; CoeffBitWidth "Coeff Bitwidth:"; mult_latency "Mult Latency"; use_hdl "Use behavioral HDL for multlipliers"; use_embedded "Use embedded multipliers"
      mask init:
      | last_tap_real_init(gcb,...
      |     'BitWidthIn', BitWidthIn,...
      |     'CoeffBitWidth', CoeffBitWidth,...
      |     'mult_latency', mult_latency,...
      |     'use_hdl', use_hdl,...
      |     'use_embedded', use_embedded);
      mask Callback use_hdl:
      | use_hdl = get_param(gcb,'use_hdl');
      | if( strcmp(use_hdl,'on')),
      |     set_param(gcb, 'use_embedded','off');
      |     set_param(gcb, 'MaskVisibilities',{'on','on','on','on','off'});
      | else,
      |     set_param(gcb, 'MaskVisibilities',{'on','on','on','on','on'});
      | end
  pol1_in1_last_tap15 : Subsystem  AncestorBlock=casper_library_pfbs/last_tap_real  mask(last_tap_real){BitWidthIn=16, CoeffBitWidth=16, mult_latency=2, use_hdl=on, use_embedded=off}
      mask prompts: BitWidthIn "Input Bitwidth:"; CoeffBitWidth "Coeff Bitwidth:"; mult_latency "Mult Latency"; use_hdl "Use behavioral HDL for multlipliers"; use_embedded "Use embedded multipliers"
      mask init:
      | last_tap_real_init(gcb,...
      |     'BitWidthIn', BitWidthIn,...
      |     'CoeffBitWidth', CoeffBitWidth,...
      |     'mult_latency', mult_latency,...
      |     'use_hdl', use_hdl,...
      |     'use_embedded', use_embedded);
      mask Callback use_hdl:
      | use_hdl = get_param(gcb,'use_hdl');
      | if( strcmp(use_hdl,'on')),
      |     set_param(gcb, 'use_embedded','off');
      |     set_param(gcb, 'MaskVisibilities',{'on','on','on','on','off'});
      | else,
      |     set_param(gcb, 'MaskVisibilities',{'on','on','on','on','on'});
      | end
  pol1_in1_last_tap2 : Subsystem  AncestorBlock=casper_library_pfbs/last_tap_real  mask(last_tap_real){BitWidthIn=16, CoeffBitWidth=16, mult_latency=2, use_hdl=on, use_embedded=off}
      mask prompts: BitWidthIn "Input Bitwidth:"; CoeffBitWidth "Coeff Bitwidth:"; mult_latency "Mult Latency"; use_hdl "Use behavioral HDL for multlipliers"; use_embedded "Use embedded multipliers"
      mask init:
      | last_tap_real_init(gcb,...
      |     'BitWidthIn', BitWidthIn,...
      |     'CoeffBitWidth', CoeffBitWidth,...
      |     'mult_latency', mult_latency,...
      |     'use_hdl', use_hdl,...
      |     'use_embedded', use_embedded);
      mask Callback use_hdl:
      | use_hdl = get_param(gcb,'use_hdl');
      | if( strcmp(use_hdl,'on')),
      |     set_param(gcb, 'use_embedded','off');
      |     set_param(gcb, 'MaskVisibilities',{'on','on','on','on','off'});
      | else,
      |     set_param(gcb, 'MaskVisibilities',{'on','on','on','on','on'});
      | end
  pol1_in1_last_tap3 : Subsystem  AncestorBlock=casper_library_pfbs/last_tap_real  mask(last_tap_real){BitWidthIn=16, CoeffBitWidth=16, mult_latency=2, use_hdl=on, use_embedded=off}
      mask prompts: BitWidthIn "Input Bitwidth:"; CoeffBitWidth "Coeff Bitwidth:"; mult_latency "Mult Latency"; use_hdl "Use behavioral HDL for multlipliers"; use_embedded "Use embedded multipliers"
      mask init:
      | last_tap_real_init(gcb,...
      |     'BitWidthIn', BitWidthIn,...
      |     'CoeffBitWidth', CoeffBitWidth,...
      |     'mult_latency', mult_latency,...
      |     'use_hdl', use_hdl,...
      |     'use_embedded', use_embedded);
      mask Callback use_hdl:
      | use_hdl = get_param(gcb,'use_hdl');
      | if( strcmp(use_hdl,'on')),
      |     set_param(gcb, 'use_embedded','off');
      |     set_param(gcb, 'MaskVisibilities',{'on','on','on','on','off'});
      | else,
      |     set_param(gcb, 'MaskVisibilities',{'on','on','on','on','on'});
      | end
  pol1_in1_last_tap4 : Subsystem  AncestorBlock=casper_library_pfbs/last_tap_real  mask(last_tap_real){BitWidthIn=16, CoeffBitWidth=16, mult_latency=2, use_hdl=on, use_embedded=off}
      mask prompts: BitWidthIn "Input Bitwidth:"; CoeffBitWidth "Coeff Bitwidth:"; mult_latency "Mult Latency"; use_hdl "Use behavioral HDL for multlipliers"; use_embedded "Use embedded multipliers"
      mask init:
      | last_tap_real_init(gcb,...
      |     'BitWidthIn', BitWidthIn,...
      |     'CoeffBitWidth', CoeffBitWidth,...
      |     'mult_latency', mult_latency,...
      |     'use_hdl', use_hdl,...
      |     'use_embedded', use_embedded);
      mask Callback use_hdl:
      | use_hdl = get_param(gcb,'use_hdl');
      | if( strcmp(use_hdl,'on')),
      |     set_param(gcb, 'use_embedded','off');
      |     set_param(gcb, 'MaskVisibilities',{'on','on','on','on','off'});
      | else,
      |     set_param(gcb, 'MaskVisibilities',{'on','on','on','on','on'});
      | end
  pol1_in1_last_tap5 : Subsystem  AncestorBlock=casper_library_pfbs/last_tap_real  mask(last_tap_real){BitWidthIn=16, CoeffBitWidth=16, mult_latency=2, use_hdl=on, use_embedded=off}
      mask prompts: BitWidthIn "Input Bitwidth:"; CoeffBitWidth "Coeff Bitwidth:"; mult_latency "Mult Latency"; use_hdl "Use behavioral HDL for multlipliers"; use_embedded "Use embedded multipliers"
      mask init:
      | last_tap_real_init(gcb,...
      |     'BitWidthIn', BitWidthIn,...
      |     'CoeffBitWidth', CoeffBitWidth,...
      |     'mult_latency', mult_latency,...
      |     'use_hdl', use_hdl,...
      |     'use_embedded', use_embedded);
      mask Callback use_hdl:
      | use_hdl = get_param(gcb,'use_hdl');
      | if( strcmp(use_hdl,'on')),
      |     set_param(gcb, 'use_embedded','off');
      |     set_param(gcb, 'MaskVisibilities',{'on','on','on','on','off'});
      | else,
      |     set_param(gcb, 'MaskVisibilities',{'on','on','on','on','on'});
      | end
  pol1_in1_last_tap6 : Subsystem  AncestorBlock=casper_library_pfbs/last_tap_real  mask(last_tap_real){BitWidthIn=16, CoeffBitWidth=16, mult_latency=2, use_hdl=on, use_embedded=off}
      mask prompts: BitWidthIn "Input Bitwidth:"; CoeffBitWidth "Coeff Bitwidth:"; mult_latency "Mult Latency"; use_hdl "Use behavioral HDL for multlipliers"; use_embedded "Use embedded multipliers"
      mask init:
      | last_tap_real_init(gcb,...
      |     'BitWidthIn', BitWidthIn,...
      |     'CoeffBitWidth', CoeffBitWidth,...
      |     'mult_latency', mult_latency,...
      |     'use_hdl', use_hdl,...
      |     'use_embedded', use_embedded);
      mask Callback use_hdl:
      | use_hdl = get_param(gcb,'use_hdl');
      | if( strcmp(use_hdl,'on')),
      |     set_param(gcb, 'use_embedded','off');
      |     set_param(gcb, 'MaskVisibilities',{'on','on','on','on','off'});
      | else,
      |     set_param(gcb, 'MaskVisibilities',{'on','on','on','on','on'});
      | end
  pol1_in1_last_tap7 : Subsystem  AncestorBlock=casper_library_pfbs/last_tap_real  mask(last_tap_real){BitWidthIn=16, CoeffBitWidth=16, mult_latency=2, use_hdl=on, use_embedded=off}
      mask prompts: BitWidthIn "Input Bitwidth:"; CoeffBitWidth "Coeff Bitwidth:"; mult_latency "Mult Latency"; use_hdl "Use behavioral HDL for multlipliers"; use_embedded "Use embedded multipliers"
      mask init:
      | last_tap_real_init(gcb,...
      |     'BitWidthIn', BitWidthIn,...
      |     'CoeffBitWidth', CoeffBitWidth,...
      |     'mult_latency', mult_latency,...
      |     'use_hdl', use_hdl,...
      |     'use_embedded', use_embedded);
      mask Callback use_hdl:
      | use_hdl = get_param(gcb,'use_hdl');
      | if( strcmp(use_hdl,'on')),
      |     set_param(gcb, 'use_embedded','off');
      |     set_param(gcb, 'MaskVisibilities',{'on','on','on','on','off'});
      | else,
      |     set_param(gcb, 'MaskVisibilities',{'on','on','on','on','on'});
      | end
  pol1_in1_last_tap8 : Subsystem  AncestorBlock=casper_library_pfbs/last_tap_real  mask(last_tap_real){BitWidthIn=16, CoeffBitWidth=16, mult_latency=2, use_hdl=on, use_embedded=off}
      mask prompts: BitWidthIn "Input Bitwidth:"; CoeffBitWidth "Coeff Bitwidth:"; mult_latency "Mult Latency"; use_hdl "Use behavioral HDL for multlipliers"; use_embedded "Use embedded multipliers"
      mask init:
      | last_tap_real_init(gcb,...
      |     'BitWidthIn', BitWidthIn,...
      |     'CoeffBitWidth', CoeffBitWidth,...
      |     'mult_latency', mult_latency,...
      |     'use_hdl', use_hdl,...
      |     'use_embedded', use_embedded);
      mask Callback use_hdl:
      | use_hdl = get_param(gcb,'use_hdl');
      | if( strcmp(use_hdl,'on')),
      |     set_param(gcb, 'use_embedded','off');
      |     set_param(gcb, 'MaskVisibilities',{'on','on','on','on','off'});
      | else,
      |     set_param(gcb, 'MaskVisibilities',{'on','on','on','on','on'});
      | end
  pol1_in1_last_tap9 : Subsystem  AncestorBlock=casper_library_pfbs/last_tap_real  mask(last_tap_real){BitWidthIn=16, CoeffBitWidth=16, mult_latency=2, use_hdl=on, use_embedded=off}
      mask prompts: BitWidthIn "Input Bitwidth:"; CoeffBitWidth "Coeff Bitwidth:"; mult_latency "Mult Latency"; use_hdl "Use behavioral HDL for multlipliers"; use_embedded "Use embedded multipliers"
      mask init:
      | last_tap_real_init(gcb,...
      |     'BitWidthIn', BitWidthIn,...
      |     'CoeffBitWidth', CoeffBitWidth,...
      |     'mult_latency', mult_latency,...
      |     'use_hdl', use_hdl,...
      |     'use_embedded', use_embedded);
      mask Callback use_hdl:
      | use_hdl = get_param(gcb,'use_hdl');
      | if( strcmp(use_hdl,'on')),
      |     set_param(gcb, 'use_embedded','off');
      |     set_param(gcb, 'MaskVisibilities',{'on','on','on','on','off'});
      | else,
      |     set_param(gcb, 'MaskVisibilities',{'on','on','on','on','on'});
      | end
  pol1_in1_tap1 : Subsystem  AncestorBlock=casper_library_pfbs/tap_real  mask(pfb_tap_real){mult_latency=2, coeff_width=16, coeff_frac_width=15, delay=16, data_width=16, bram_latency=2, use_hdl=on, use_embedded=off}
      mask prompts: mult_latency "Multiplier Latency"; coeff_width "Coefficient Bit Width In"; coeff_frac_width "Coefficient Fractional Bits"; delay "Data/Sync Delay"; data_width "Data Bit Width In"; bram_latency "BRAM Latency"; use_hdl "Use behavioral HDL for multlipliers"; use_embedded "Use embedded multipliers"
      mask init:
      | use_hdl = get_param(gcb,'use_hdl');
      | use_embedded = get_param(gcb,'use_embedded');
      | set_param(gcb,'LinkStatus','inactive');
      | 
      | set_param([gcb,'/Mult'],'use_embedded',use_embedded);
      | set_param([gcb,'/Mult'],'use_behavioral_HDL',use_hdl);
  pol1_in1_tap10 : Subsystem  AncestorBlock=casper_library_pfbs/tap_real  mask(pfb_tap_real){mult_latency=2, coeff_width=16, coeff_frac_width=15, delay=16, data_width=16, bram_latency=2, use_hdl=on, use_embedded=off}
      mask prompts: mult_latency "Multiplier Latency"; coeff_width "Coefficient Bit Width In"; coeff_frac_width "Coefficient Fractional Bits"; delay "Data/Sync Delay"; data_width "Data Bit Width In"; bram_latency "BRAM Latency"; use_hdl "Use behavioral HDL for multlipliers"; use_embedded "Use embedded multipliers"
      mask init: same as rfsoc4x2_ospfb_128/pfb_fir_real7/pol1_in1_tap1
  pol1_in1_tap11 : Subsystem  AncestorBlock=casper_library_pfbs/tap_real  mask(pfb_tap_real){mult_latency=2, coeff_width=16, coeff_frac_width=15, delay=16, data_width=16, bram_latency=2, use_hdl=on, use_embedded=off}
      mask prompts: mult_latency "Multiplier Latency"; coeff_width "Coefficient Bit Width In"; coeff_frac_width "Coefficient Fractional Bits"; delay "Data/Sync Delay"; data_width "Data Bit Width In"; bram_latency "BRAM Latency"; use_hdl "Use behavioral HDL for multlipliers"; use_embedded "Use embedded multipliers"
      mask init: same as rfsoc4x2_ospfb_128/pfb_fir_real7/pol1_in1_tap1
  pol1_in1_tap12 : Subsystem  AncestorBlock=casper_library_pfbs/tap_real  mask(pfb_tap_real){mult_latency=2, coeff_width=16, coeff_frac_width=15, delay=16, data_width=16, bram_latency=2, use_hdl=on, use_embedded=off}
      mask prompts: mult_latency "Multiplier Latency"; coeff_width "Coefficient Bit Width In"; coeff_frac_width "Coefficient Fractional Bits"; delay "Data/Sync Delay"; data_width "Data Bit Width In"; bram_latency "BRAM Latency"; use_hdl "Use behavioral HDL for multlipliers"; use_embedded "Use embedded multipliers"
      mask init: same as rfsoc4x2_ospfb_128/pfb_fir_real7/pol1_in1_tap1
  pol1_in1_tap13 : Subsystem  AncestorBlock=casper_library_pfbs/tap_real  mask(pfb_tap_real){mult_latency=2, coeff_width=16, coeff_frac_width=15, delay=16, data_width=16, bram_latency=2, use_hdl=on, use_embedded=off}
      mask prompts: mult_latency "Multiplier Latency"; coeff_width "Coefficient Bit Width In"; coeff_frac_width "Coefficient Fractional Bits"; delay "Data/Sync Delay"; data_width "Data Bit Width In"; bram_latency "BRAM Latency"; use_hdl "Use behavioral HDL for multlipliers"; use_embedded "Use embedded multipliers"
      mask init: same as rfsoc4x2_ospfb_128/pfb_fir_real7/pol1_in1_tap1
  pol1_in1_tap14 : Subsystem  AncestorBlock=casper_library_pfbs/tap_real  mask(pfb_tap_real){mult_latency=2, coeff_width=16, coeff_frac_width=15, delay=16, data_width=16, bram_latency=2, use_hdl=on, use_embedded=off}
      mask prompts: mult_latency "Multiplier Latency"; coeff_width "Coefficient Bit Width In"; coeff_frac_width "Coefficient Fractional Bits"; delay "Data/Sync Delay"; data_width "Data Bit Width In"; bram_latency "BRAM Latency"; use_hdl "Use behavioral HDL for multlipliers"; use_embedded "Use embedded multipliers"
      mask init: same as rfsoc4x2_ospfb_128/pfb_fir_real7/pol1_in1_tap1
  pol1_in1_tap15 : Subsystem  AncestorBlock=casper_library_pfbs/tap_real  mask(pfb_tap_real){mult_latency=2, coeff_width=16, coeff_frac_width=15, delay=16, data_width=16, bram_latency=2, use_hdl=on, use_embedded=off}
      mask prompts: mult_latency "Multiplier Latency"; coeff_width "Coefficient Bit Width In"; coeff_frac_width "Coefficient Fractional Bits"; delay "Data/Sync Delay"; data_width "Data Bit Width In"; bram_latency "BRAM Latency"; use_hdl "Use behavioral HDL for multlipliers"; use_embedded "Use embedded multipliers"
      mask init: same as rfsoc4x2_ospfb_128/pfb_fir_real7/pol1_in1_tap1
  pol1_in1_tap16 : Subsystem  AncestorBlock=casper_library_pfbs/tap_real  mask(pfb_tap_real){mult_latency=2, coeff_width=16, coeff_frac_width=15, delay=16, data_width=16, bram_latency=2, use_hdl=on, use_embedded=off}
      mask prompts: mult_latency "Multiplier Latency"; coeff_width "Coefficient Bit Width In"; coeff_frac_width "Coefficient Fractional Bits"; delay "Data/Sync Delay"; data_width "Data Bit Width In"; bram_latency "BRAM Latency"; use_hdl "Use behavioral HDL for multlipliers"; use_embedded "Use embedded multipliers"
      mask init: same as rfsoc4x2_ospfb_128/pfb_fir_real7/pol1_in1_tap1
  pol1_in1_tap17 : Subsystem  AncestorBlock=casper_library_pfbs/tap_real  mask(pfb_tap_real){mult_latency=2, coeff_width=16, coeff_frac_width=15, delay=16, data_width=16, bram_latency=2, use_hdl=on, use_embedded=off}
      mask prompts: mult_latency "Multiplier Latency"; coeff_width "Coefficient Bit Width In"; coeff_frac_width "Coefficient Fractional Bits"; delay "Data/Sync Delay"; data_width "Data Bit Width In"; bram_latency "BRAM Latency"; use_hdl "Use behavioral HDL for multlipliers"; use_embedded "Use embedded multipliers"
      mask init: same as rfsoc4x2_ospfb_128/pfb_fir_real7/pol1_in1_tap1
  pol1_in1_tap18 : Subsystem  AncestorBlock=casper_library_pfbs/tap_real  mask(pfb_tap_real){mult_latency=2, coeff_width=16, coeff_frac_width=15, delay=16, data_width=16, bram_latency=2, use_hdl=on, use_embedded=off}
      mask prompts: mult_latency "Multiplier Latency"; coeff_width "Coefficient Bit Width In"; coeff_frac_width "Coefficient Fractional Bits"; delay "Data/Sync Delay"; data_width "Data Bit Width In"; bram_latency "BRAM Latency"; use_hdl "Use behavioral HDL for multlipliers"; use_embedded "Use embedded multipliers"
      mask init: same as rfsoc4x2_ospfb_128/pfb_fir_real7/pol1_in1_tap1
  pol1_in1_tap19 : Subsystem  AncestorBlock=casper_library_pfbs/tap_real  mask(pfb_tap_real){mult_latency=2, coeff_width=16, coeff_frac_width=15, delay=16, data_width=16, bram_latency=2, use_hdl=on, use_embedded=off}
      mask prompts: mult_latency "Multiplier Latency"; coeff_width "Coefficient Bit Width In"; coeff_frac_width "Coefficient Fractional Bits"; delay "Data/Sync Delay"; data_width "Data Bit Width In"; bram_latency "BRAM Latency"; use_hdl "Use behavioral HDL for multlipliers"; use_embedded "Use embedded multipliers"
      mask init: same as rfsoc4x2_ospfb_128/pfb_fir_real7/pol1_in1_tap1
  pol1_in1_tap2 : Subsystem  AncestorBlock=casper_library_pfbs/tap_real  mask(pfb_tap_real){mult_latency=2, coeff_width=16, coeff_frac_width=15, delay=16, data_width=16, bram_latency=2, use_hdl=on, use_embedded=off}
      mask prompts: mult_latency "Multiplier Latency"; coeff_width "Coefficient Bit Width In"; coeff_frac_width "Coefficient Fractional Bits"; delay "Data/Sync Delay"; data_width "Data Bit Width In"; bram_latency "BRAM Latency"; use_hdl "Use behavioral HDL for multlipliers"; use_embedded "Use embedded multipliers"
      mask init: same as rfsoc4x2_ospfb_128/pfb_fir_real7/pol1_in1_tap1
  pol1_in1_tap20 : Subsystem  AncestorBlock=casper_library_pfbs/tap_real  mask(pfb_tap_real){mult_latency=2, coeff_width=16, coeff_frac_width=15, delay=16, data_width=16, bram_latency=2, use_hdl=on, use_embedded=off}
      mask prompts: mult_latency "Multiplier Latency"; coeff_width "Coefficient Bit Width In"; coeff_frac_width "Coefficient Fractional Bits"; delay "Data/Sync Delay"; data_width "Data Bit Width In"; bram_latency "BRAM Latency"; use_hdl "Use behavioral HDL for multlipliers"; use_embedded "Use embedded multipliers"
      mask init: same as rfsoc4x2_ospfb_128/pfb_fir_real7/pol1_in1_tap1
  pol1_in1_tap21 : Subsystem  AncestorBlock=casper_library_pfbs/tap_real  mask(pfb_tap_real){mult_latency=2, coeff_width=16, coeff_frac_width=15, delay=16, data_width=16, bram_latency=2, use_hdl=on, use_embedded=off}
      mask prompts: mult_latency "Multiplier Latency"; coeff_width "Coefficient Bit Width In"; coeff_frac_width "Coefficient Fractional Bits"; delay "Data/Sync Delay"; data_width "Data Bit Width In"; bram_latency "BRAM Latency"; use_hdl "Use behavioral HDL for multlipliers"; use_embedded "Use embedded multipliers"
      mask init: same as rfsoc4x2_ospfb_128/pfb_fir_real7/pol1_in1_tap1
  pol1_in1_tap22 : Subsystem  AncestorBlock=casper_library_pfbs/tap_real  mask(pfb_tap_real){mult_latency=2, coeff_width=16, coeff_frac_width=15, delay=16, data_width=16, bram_latency=2, use_hdl=on, use_embedded=off}
      mask prompts: mult_latency "Multiplier Latency"; coeff_width "Coefficient Bit Width In"; coeff_frac_width "Coefficient Fractional Bits"; delay "Data/Sync Delay"; data_width "Data Bit Width In"; bram_latency "BRAM Latency"; use_hdl "Use behavioral HDL for multlipliers"; use_embedded "Use embedded multipliers"
      mask init: same as rfsoc4x2_ospfb_128/pfb_fir_real7/pol1_in1_tap1
  pol1_in1_tap23 : Subsystem  AncestorBlock=casper_library_pfbs/tap_real  mask(pfb_tap_real){mult_latency=2, coeff_width=16, coeff_frac_width=15, delay=16, data_width=16, bram_latency=2, use_hdl=on, use_embedded=off}
      mask prompts: mult_latency "Multiplier Latency"; coeff_width "Coefficient Bit Width In"; coeff_frac_width "Coefficient Fractional Bits"; delay "Data/Sync Delay"; data_width "Data Bit Width In"; bram_latency "BRAM Latency"; use_hdl "Use behavioral HDL for multlipliers"; use_embedded "Use embedded multipliers"
      mask init: same as rfsoc4x2_ospfb_128/pfb_fir_real7/pol1_in1_tap1
  pol1_in1_tap24 : Subsystem  AncestorBlock=casper_library_pfbs/tap_real  mask(pfb_tap_real){mult_latency=2, coeff_width=16, coeff_frac_width=15, delay=16, data_width=16, bram_latency=2, use_hdl=on, use_embedded=off}
      mask prompts: mult_latency "Multiplier Latency"; coeff_width "Coefficient Bit Width In"; coeff_frac_width "Coefficient Fractional Bits"; delay "Data/Sync Delay"; data_width "Data Bit Width In"; bram_latency "BRAM Latency"; use_hdl "Use behavioral HDL for multlipliers"; use_embedded "Use embedded multipliers"
      mask init: same as rfsoc4x2_ospfb_128/pfb_fir_real7/pol1_in1_tap1
  pol1_in1_tap25 : Subsystem  AncestorBlock=casper_library_pfbs/tap_real  mask(pfb_tap_real){mult_latency=2, coeff_width=16, coeff_frac_width=15, delay=16, data_width=16, bram_latency=2, use_hdl=on, use_embedded=off}
      mask prompts: mult_latency "Multiplier Latency"; coeff_width "Coefficient Bit Width In"; coeff_frac_width "Coefficient Fractional Bits"; delay "Data/Sync Delay"; data_width "Data Bit Width In"; bram_latency "BRAM Latency"; use_hdl "Use behavioral HDL for multlipliers"; use_embedded "Use embedded multipliers"
      mask init: same as rfsoc4x2_ospfb_128/pfb_fir_real7/pol1_in1_tap1
  pol1_in1_tap26 : Subsystem  AncestorBlock=casper_library_pfbs/tap_real  mask(pfb_tap_real){mult_latency=2, coeff_width=16, coeff_frac_width=15, delay=16, data_width=16, bram_latency=2, use_hdl=on, use_embedded=off}
      mask prompts: mult_latency "Multiplier Latency"; coeff_width "Coefficient Bit Width In"; coeff_frac_width "Coefficient Fractional Bits"; delay "Data/Sync Delay"; data_width "Data Bit Width In"; bram_latency "BRAM Latency"; use_hdl "Use behavioral HDL for multlipliers"; use_embedded "Use embedded multipliers"
      mask init: same as rfsoc4x2_ospfb_128/pfb_fir_real7/pol1_in1_tap1
  pol1_in1_tap27 : Subsystem  AncestorBlock=casper_library_pfbs/tap_real  mask(pfb_tap_real){mult_latency=2, coeff_width=16, coeff_frac_width=15, delay=16, data_width=16, bram_latency=2, use_hdl=on, use_embedded=off}
      mask prompts: mult_latency "Multiplier Latency"; coeff_width "Coefficient Bit Width In"; coeff_frac_width "Coefficient Fractional Bits"; delay "Data/Sync Delay"; data_width "Data Bit Width In"; bram_latency "BRAM Latency"; use_hdl "Use behavioral HDL for multlipliers"; use_embedded "Use embedded multipliers"
      mask init: same as rfsoc4x2_ospfb_128/pfb_fir_real7/pol1_in1_tap1
  pol1_in1_tap28 : Subsystem  AncestorBlock=casper_library_pfbs/tap_real  mask(pfb_tap_real){mult_latency=2, coeff_width=16, coeff_frac_width=15, delay=16, data_width=16, bram_latency=2, use_hdl=on, use_embedded=off}
      mask prompts: mult_latency "Multiplier Latency"; coeff_width "Coefficient Bit Width In"; coeff_frac_width "Coefficient Fractional Bits"; delay "Data/Sync Delay"; data_width "Data Bit Width In"; bram_latency "BRAM Latency"; use_hdl "Use behavioral HDL for multlipliers"; use_embedded "Use embedded multipliers"
      mask init: same as rfsoc4x2_ospfb_128/pfb_fir_real7/pol1_in1_tap1
  pol1_in1_tap29 : Subsystem  AncestorBlock=casper_library_pfbs/tap_real  mask(pfb_tap_real){mult_latency=2, coeff_width=16, coeff_frac_width=15, delay=16, data_width=16, bram_latency=2, use_hdl=on, use_embedded=off}
      mask prompts: mult_latency "Multiplier Latency"; coeff_width "Coefficient Bit Width In"; coeff_frac_width "Coefficient Fractional Bits"; delay "Data/Sync Delay"; data_width "Data Bit Width In"; bram_latency "BRAM Latency"; use_hdl "Use behavioral HDL for multlipliers"; use_embedded "Use embedded multipliers"
      mask init: same as rfsoc4x2_ospfb_128/pfb_fir_real7/pol1_in1_tap1
  pol1_in1_tap3 : Subsystem  AncestorBlock=casper_library_pfbs/tap_real  mask(pfb_tap_real){mult_latency=2, coeff_width=16, coeff_frac_width=15, delay=16, data_width=16, bram_latency=2, use_hdl=on, use_embedded=off}
      mask prompts: mult_latency "Multiplier Latency"; coeff_width "Coefficient Bit Width In"; coeff_frac_width "Coefficient Fractional Bits"; delay "Data/Sync Delay"; data_width "Data Bit Width In"; bram_latency "BRAM Latency"; use_hdl "Use behavioral HDL for multlipliers"; use_embedded "Use embedded multipliers"
      mask init: same as rfsoc4x2_ospfb_128/pfb_fir_real7/pol1_in1_tap1
  pol1_in1_tap30 : Subsystem  AncestorBlock=casper_library_pfbs/tap_real  mask(pfb_tap_real){mult_latency=2, coeff_width=16, coeff_frac_width=15, delay=16, data_width=16, bram_latency=2, use_hdl=on, use_embedded=off}
      mask prompts: mult_latency "Multiplier Latency"; coeff_width "Coefficient Bit Width In"; coeff_frac_width "Coefficient Fractional Bits"; delay "Data/Sync Delay"; data_width "Data Bit Width In"; bram_latency "BRAM Latency"; use_hdl "Use behavioral HDL for multlipliers"; use_embedded "Use embedded multipliers"
      mask init: same as rfsoc4x2_ospfb_128/pfb_fir_real7/pol1_in1_tap1
  pol1_in1_tap31 : Subsystem  AncestorBlock=casper_library_pfbs/tap_real  mask(pfb_tap_real){mult_latency=2, coeff_width=16, coeff_frac_width=15, delay=16, data_width=16, bram_latency=2, use_hdl=on, use_embedded=off}
      mask prompts: mult_latency "Multiplier Latency"; coeff_width "Coefficient Bit Width In"; coeff_frac_width "Coefficient Fractional Bits"; delay "Data/Sync Delay"; data_width "Data Bit Width In"; bram_latency "BRAM Latency"; use_hdl "Use behavioral HDL for multlipliers"; use_embedded "Use embedded multipliers"
      mask init: same as rfsoc4x2_ospfb_128/pfb_fir_real7/pol1_in1_tap1
  pol1_in1_tap32 : Subsystem  AncestorBlock=casper_library_pfbs/tap_real  mask(pfb_tap_real){mult_latency=2, coeff_width=16, coeff_frac_width=15, delay=16, data_width=16, bram_latency=2, use_hdl=on, use_embedded=off}
      mask prompts: mult_latency "Multiplier Latency"; coeff_width "Coefficient Bit Width In"; coeff_frac_width "Coefficient Fractional Bits"; delay "Data/Sync Delay"; data_width "Data Bit Width In"; bram_latency "BRAM Latency"; use_hdl "Use behavioral HDL for multlipliers"; use_embedded "Use embedded multipliers"
      mask init: same as rfsoc4x2_ospfb_128/pfb_fir_real7/pol1_in1_tap1
  pol1_in1_tap4 : Subsystem  AncestorBlock=casper_library_pfbs/tap_real  mask(pfb_tap_real){mult_latency=2, coeff_width=16, coeff_frac_width=15, delay=16, data_width=16, bram_latency=2, use_hdl=on, use_embedded=off}
      mask prompts: mult_latency "Multiplier Latency"; coeff_width "Coefficient Bit Width In"; coeff_frac_width "Coefficient Fractional Bits"; delay "Data/Sync Delay"; data_width "Data Bit Width In"; bram_latency "BRAM Latency"; use_hdl "Use behavioral HDL for multlipliers"; use_embedded "Use embedded multipliers"
      mask init: same as rfsoc4x2_ospfb_128/pfb_fir_real7/pol1_in1_tap1
  pol1_in1_tap5 : Subsystem  AncestorBlock=casper_library_pfbs/tap_real  mask(pfb_tap_real){mult_latency=2, coeff_width=16, coeff_frac_width=15, delay=16, data_width=16, bram_latency=2, use_hdl=on, use_embedded=off}
      mask prompts: mult_latency "Multiplier Latency"; coeff_width "Coefficient Bit Width In"; coeff_frac_width "Coefficient Fractional Bits"; delay "Data/Sync Delay"; data_width "Data Bit Width In"; bram_latency "BRAM Latency"; use_hdl "Use behavioral HDL for multlipliers"; use_embedded "Use embedded multipliers"
      mask init: same as rfsoc4x2_ospfb_128/pfb_fir_real7/pol1_in1_tap1
  pol1_in1_tap6 : Subsystem  AncestorBlock=casper_library_pfbs/tap_real  mask(pfb_tap_real){mult_latency=2, coeff_width=16, coeff_frac_width=15, delay=16, data_width=16, bram_latency=2, use_hdl=on, use_embedded=off}
      mask prompts: mult_latency "Multiplier Latency"; coeff_width "Coefficient Bit Width In"; coeff_frac_width "Coefficient Fractional Bits"; delay "Data/Sync Delay"; data_width "Data Bit Width In"; bram_latency "BRAM Latency"; use_hdl "Use behavioral HDL for multlipliers"; use_embedded "Use embedded multipliers"
      mask init: same as rfsoc4x2_ospfb_128/pfb_fir_real7/pol1_in1_tap1
  pol1_in1_tap7 : Subsystem  AncestorBlock=casper_library_pfbs/tap_real  mask(pfb_tap_real){mult_latency=2, coeff_width=16, coeff_frac_width=15, delay=16, data_width=16, bram_latency=2, use_hdl=on, use_embedded=off}
      mask prompts: mult_latency "Multiplier Latency"; coeff_width "Coefficient Bit Width In"; coeff_frac_width "Coefficient Fractional Bits"; delay "Data/Sync Delay"; data_width "Data Bit Width In"; bram_latency "BRAM Latency"; use_hdl "Use behavioral HDL for multlipliers"; use_embedded "Use embedded multipliers"
      mask init: same as rfsoc4x2_ospfb_128/pfb_fir_real7/pol1_in1_tap1
  pol1_in1_tap8 : Subsystem  AncestorBlock=casper_library_pfbs/tap_real  mask(pfb_tap_real){mult_latency=2, coeff_width=16, coeff_frac_width=15, delay=16, data_width=16, bram_latency=2, use_hdl=on, use_embedded=off}
      mask prompts: mult_latency "Multiplier Latency"; coeff_width "Coefficient Bit Width In"; coeff_frac_width "Coefficient Fractional Bits"; delay "Data/Sync Delay"; data_width "Data Bit Width In"; bram_latency "BRAM Latency"; use_hdl "Use behavioral HDL for multlipliers"; use_embedded "Use embedded multipliers"
      mask init: same as rfsoc4x2_ospfb_128/pfb_fir_real7/pol1_in1_tap1
  pol1_in1_tap9 : Subsystem  AncestorBlock=casper_library_pfbs/tap_real  mask(pfb_tap_real){mult_latency=2, coeff_width=16, coeff_frac_width=15, delay=16, data_width=16, bram_latency=2, use_hdl=on, use_embedded=off}
      mask prompts: mult_latency "Multiplier Latency"; coeff_width "Coefficient Bit Width In"; coeff_frac_width "Coefficient Fractional Bits"; delay "Data/Sync Delay"; data_width "Data Bit Width In"; bram_latency "BRAM Latency"; use_hdl "Use behavioral HDL for multlipliers"; use_embedded "Use embedded multipliers"
      mask init: same as rfsoc4x2_ospfb_128/pfb_fir_real7/pol1_in1_tap1
  pol1_in2_coeffs : Subsystem  AncestorBlock=casper_library_pfbs/pfb_coeff_gen  mask(pfb_coeff_gen){PFBSize=8, CoeffBitWidth=16, TotalTaps=4, CoeffDistMem=off, WindowType=hamming, bram_latency=2, n_inputs=4, nput=1, fwidth=2, debug_mode=off, fan_latency=1}
      mask prompts: PFBSize "Size of PFB: (2^? pnts)"; CoeffBitWidth "Bitwidth of Coefficients:"; TotalTaps "Total Number of Taps:"; CoeffDistMem "Implement Coeff Gen in Distributed Memory"; WindowType "Windowing Function:"; bram_latency "BRAM Latency"; n_inputs "Number of Simultaneous Inputs: (2^?)"; nput "This is input number:"; fwidth "Bin Width (normal=1)"; debug_mode "Debug mode - coeffs are a [1:pfb_size*taps] ramp."; fan_latency "Fanout latency"
      mask init: same as rfsoc4x2_ospfb_128/pfb_fir_real7/pol1_in10_coeffs
      settings: AttributesFormatString=|
      | PFBSize=8, n_inputs=4,
      | taps=4, input=1
  pol1_in3_coeffs : Subsystem  AncestorBlock=casper_library_pfbs/pfb_coeff_gen  mask(pfb_coeff_gen){PFBSize=8, CoeffBitWidth=16, TotalTaps=4, CoeffDistMem=off, WindowType=hamming, bram_latency=2, n_inputs=4, nput=2, fwidth=2, debug_mode=off, fan_latency=1}
      mask prompts: PFBSize "Size of PFB: (2^? pnts)"; CoeffBitWidth "Bitwidth of Coefficients:"; TotalTaps "Total Number of Taps:"; CoeffDistMem "Implement Coeff Gen in Distributed Memory"; WindowType "Windowing Function:"; bram_latency "BRAM Latency"; n_inputs "Number of Simultaneous Inputs: (2^?)"; nput "This is input number:"; fwidth "Bin Width (normal=1)"; debug_mode "Debug mode - coeffs are a [1:pfb_size*taps] ramp."; fan_latency "Fanout latency"
      mask init: same as rfsoc4x2_ospfb_128/pfb_fir_real7/pol1_in10_coeffs
      settings: AttributesFormatString=|
      | PFBSize=8, n_inputs=4,
      | taps=4, input=2
  pol1_in4_coeffs : Subsystem  AncestorBlock=casper_library_pfbs/pfb_coeff_gen  mask(pfb_coeff_gen){PFBSize=8, CoeffBitWidth=16, TotalTaps=4, CoeffDistMem=off, WindowType=hamming, bram_latency=2, n_inputs=4, nput=3, fwidth=2, debug_mode=off, fan_latency=1}
      mask prompts: PFBSize "Size of PFB: (2^? pnts)"; CoeffBitWidth "Bitwidth of Coefficients:"; TotalTaps "Total Number of Taps:"; CoeffDistMem "Implement Coeff Gen in Distributed Memory"; WindowType "Windowing Function:"; bram_latency "BRAM Latency"; n_inputs "Number of Simultaneous Inputs: (2^?)"; nput "This is input number:"; fwidth "Bin Width (normal=1)"; debug_mode "Debug mode - coeffs are a [1:pfb_size*taps] ramp."; fan_latency "Fanout latency"
      mask init: same as rfsoc4x2_ospfb_128/pfb_fir_real7/pol1_in10_coeffs
      settings: AttributesFormatString=|
      | PFBSize=8, n_inputs=4,
      | taps=4, input=3
  pol1_in5_coeffs : Subsystem  AncestorBlock=casper_library_pfbs/pfb_coeff_gen  mask(pfb_coeff_gen){PFBSize=8, CoeffBitWidth=16, TotalTaps=4, CoeffDistMem=off, WindowType=hamming, bram_latency=2, n_inputs=4, nput=4, fwidth=2, debug_mode=off, fan_latency=1}
      mask prompts: PFBSize "Size of PFB: (2^? pnts)"; CoeffBitWidth "Bitwidth of Coefficients:"; TotalTaps "Total Number of Taps:"; CoeffDistMem "Implement Coeff Gen in Distributed Memory"; WindowType "Windowing Function:"; bram_latency "BRAM Latency"; n_inputs "Number of Simultaneous Inputs: (2^?)"; nput "This is input number:"; fwidth "Bin Width (normal=1)"; debug_mode "Debug mode - coeffs are a [1:pfb_size*taps] ramp."; fan_latency "Fanout latency"
      mask init: same as rfsoc4x2_ospfb_128/pfb_fir_real7/pol1_in10_coeffs
      settings: AttributesFormatString=|
      | PFBSize=8, n_inputs=4,
      | taps=4, input=4
  pol1_in6_coeffs : Subsystem  AncestorBlock=casper_library_pfbs/pfb_coeff_gen  mask(pfb_coeff_gen){PFBSize=8, CoeffBitWidth=16, TotalTaps=4, CoeffDistMem=off, WindowType=hamming, bram_latency=2, n_inputs=4, nput=5, fwidth=2, debug_mode=off, fan_latency=1}
      mask prompts: PFBSize "Size of PFB: (2^? pnts)"; CoeffBitWidth "Bitwidth of Coefficients:"; TotalTaps "Total Number of Taps:"; CoeffDistMem "Implement Coeff Gen in Distributed Memory"; WindowType "Windowing Function:"; bram_latency "BRAM Latency"; n_inputs "Number of Simultaneous Inputs: (2^?)"; nput "This is input number:"; fwidth "Bin Width (normal=1)"; debug_mode "Debug mode - coeffs are a [1:pfb_size*taps] ramp."; fan_latency "Fanout latency"
      mask init: same as rfsoc4x2_ospfb_128/pfb_fir_real7/pol1_in10_coeffs
      settings: AttributesFormatString=|
      | PFBSize=8, n_inputs=4,
      | taps=4, input=5
  pol1_in7_coeffs : Subsystem  AncestorBlock=casper_library_pfbs/pfb_coeff_gen  mask(pfb_coeff_gen){PFBSize=8, CoeffBitWidth=16, TotalTaps=4, CoeffDistMem=off, WindowType=hamming, bram_latency=2, n_inputs=4, nput=6, fwidth=2, debug_mode=off, fan_latency=1}
      mask prompts: PFBSize "Size of PFB: (2^? pnts)"; CoeffBitWidth "Bitwidth of Coefficients:"; TotalTaps "Total Number of Taps:"; CoeffDistMem "Implement Coeff Gen in Distributed Memory"; WindowType "Windowing Function:"; bram_latency "BRAM Latency"; n_inputs "Number of Simultaneous Inputs: (2^?)"; nput "This is input number:"; fwidth "Bin Width (normal=1)"; debug_mode "Debug mode - coeffs are a [1:pfb_size*taps] ramp."; fan_latency "Fanout latency"
      mask init: same as rfsoc4x2_ospfb_128/pfb_fir_real7/pol1_in10_coeffs
      settings: AttributesFormatString=|
      | PFBSize=8, n_inputs=4,
      | taps=4, input=6
  pol1_in8_coeffs : Subsystem  AncestorBlock=casper_library_pfbs/pfb_coeff_gen  mask(pfb_coeff_gen){PFBSize=8, CoeffBitWidth=16, TotalTaps=4, CoeffDistMem=off, WindowType=hamming, bram_latency=2, n_inputs=4, nput=7, fwidth=2, debug_mode=off, fan_latency=1}
      mask prompts: PFBSize "Size of PFB: (2^? pnts)"; CoeffBitWidth "Bitwidth of Coefficients:"; TotalTaps "Total Number of Taps:"; CoeffDistMem "Implement Coeff Gen in Distributed Memory"; WindowType "Windowing Function:"; bram_latency "BRAM Latency"; n_inputs "Number of Simultaneous Inputs: (2^?)"; nput "This is input number:"; fwidth "Bin Width (normal=1)"; debug_mode "Debug mode - coeffs are a [1:pfb_size*taps] ramp."; fan_latency "Fanout latency"
      mask init: same as rfsoc4x2_ospfb_128/pfb_fir_real7/pol1_in10_coeffs
      settings: AttributesFormatString=|
      | PFBSize=8, n_inputs=4,
      | taps=4, input=7
  pol1_in9_coeffs : Subsystem  AncestorBlock=casper_library_pfbs/pfb_coeff_gen  mask(pfb_coeff_gen){PFBSize=8, CoeffBitWidth=16, TotalTaps=4, CoeffDistMem=off, WindowType=hamming, bram_latency=2, n_inputs=4, nput=8, fwidth=2, debug_mode=off, fan_latency=1}
      mask prompts: PFBSize "Size of PFB: (2^? pnts)"; CoeffBitWidth "Bitwidth of Coefficients:"; TotalTaps "Total Number of Taps:"; CoeffDistMem "Implement Coeff Gen in Distributed Memory"; WindowType "Windowing Function:"; bram_latency "BRAM Latency"; n_inputs "Number of Simultaneous Inputs: (2^?)"; nput "This is input number:"; fwidth "Bin Width (normal=1)"; debug_mode "Debug mode - coeffs are a [1:pfb_size*taps] ramp."; fan_latency "Fanout latency"
      mask init: same as rfsoc4x2_ospfb_128/pfb_fir_real7/pol1_in10_coeffs
      settings: AttributesFormatString=|
      | PFBSize=8, n_inputs=4,
      | taps=4, input=8
  scale_1_{1..16} (16 alike) : xbsIndex_r4/Scale  scale_factor=-1  dbl_ovrd=off  block_type=scale
  sync_out : Outport  VectorParamsAs1DForOutWhenUnconnected=off
  pol1_out1 : Outport  Port=2  VectorParamsAs1DForOutWhenUnconnected=off
  pol1_out2 : Outport  Port=3  VectorParamsAs1DForOutWhenUnconnected=off
  pol1_out3 : Outport  Port=4
  pol1_out4 : Outport  Port=5
  pol1_out5 : Outport  Port=6
  pol1_out6 : Outport  Port=7
  pol1_out7 : Outport  Port=8
  pol1_out8 : Outport  Port=9
  pol1_out9 : Outport  Port=10
  pol1_out10 : Outport  Port=11
  pol1_out11 : Outport  Port=12
  pol1_out12 : Outport  Port=13
  pol1_out13 : Outport  Port=14
  pol1_out14 : Outport  Port=15
  pol1_out15 : Outport  Port=16
  pol1_out16 : Outport  Port=17
  wires:
  pol1_in1_tap3/1(dout) -> pol1_in1_last_tap/1(din)
  Delay1/1 -> Logical9/1
  adder_1_1/2(dout) -> scale_1_1/1
  Delay10/1 -> adder_1_1/1(sync)
  Delay/1 -> sync_out/1
  delay1/1 -> Delay/1
  convert_1_1/1 -> pol1_out1/1
  Delay6/1 -> adder_1_1/4(din3)
  Delay5/1 -> adder_1_1/3(din2)
  Delay4/1 -> adder_1_1/2(din1)
  Delay3/1 -> Delay10/1
  pol1_in1_last_tap/2(sync_out) -> Delay3/1
  pol1_in1_tap2/6(write_en_out) -> pol1_in1_tap3/5(write_en_in)
  pol1_in1_tap2/5(add_out) -> pol1_in1_tap3/4(addr_in)
  pol1_in1_first_tap/6(write_en_out) -> pol1_in1_tap2/5(write_en_in)
  pol1_in1_first_tap/5(add_out) -> pol1_in1_tap2/4(addr_in)
  [addr] -> pol1_in1_first_tap/4(addr_in)
  [tap_write_en] -> pol1_in1_first_tap/5(write_en_in)
  pol1_in1_coeffs/1(dout) -> pol1_in1_first_tap/1(din)
  Relational6/1 -> [tap_write_en]
  Counter10/1 -> Slice2/1, Relational6/1
  Constant28/1 -> Relational6/2
  AddSub2/1 -> [addr]
  edge_detect3/1(out) -> Logical9/2
  en_ctrl/1 -> Delay1/1
  Counter9/1 -> AddSub2/1
  Delay76/1 -> AddSub2/2
  Logical9/1 -> Counter9/2
  Slice2/1 -> edge_detect3/1(in)
  Delay2/1 -> Counter9/1, Counter10/1, Counter14/1
  Counter14/1 -> Delay76/1
  pol1_in1_tap3/4(taps_out) -> Delay6/1
  pol1_in1_tap3/3(coeff_out) -> pol1_in1_last_tap/3(coeff)
  pol1_in1_tap3/2(sync_out) -> pol1_in1_last_tap/2(sync)
  pol1_in1_tap2/4(taps_out) -> Delay5/1
  pol1_in1_tap2/3(coeff_out) -> pol1_in1_tap3/3(coeff)
  pol1_in1_tap2/2(sync_out) -> pol1_in1_tap3/2(sync)
  pol1_in1_tap2/1(dout) -> pol1_in1_tap3/1(din)
  pol1_in1_first_tap/4(taps_out) -> Delay4/1
  pol1_in1_first_tap/3(coeff_out) -> pol1_in1_tap2/3(coeff)
  pol1_in1_first_tap/2(sync_out) -> pol1_in1_tap2/2(sync)
  pol1_in1_first_tap/1(dout) -> pol1_in1_tap2/1(din)
  convert_1_16/1 -> pol1_out16/1
  scale_1_16/1 -> convert_1_16/1
  adder_1_16/2(dout) -> scale_1_16/1
  convert_1_15/1 -> pol1_out15/1
  scale_1_15/1 -> convert_1_15/1
  adder_1_15/2(dout) -> scale_1_15/1
  convert_1_14/1 -> pol1_out14/1
  scale_1_14/1 -> convert_1_14/1
  adder_1_14/2(dout) -> scale_1_14/1
  convert_1_13/1 -> pol1_out13/1
  scale_1_13/1 -> convert_1_13/1
  adder_1_13/2(dout) -> scale_1_13/1
  convert_1_12/1 -> pol1_out12/1
  scale_1_12/1 -> convert_1_12/1
  adder_1_12/2(dout) -> scale_1_12/1
  convert_1_11/1 -> pol1_out11/1
  scale_1_11/1 -> convert_1_11/1
  adder_1_11/2(dout) -> scale_1_11/1
  convert_1_10/1 -> pol1_out10/1
  scale_1_10/1 -> convert_1_10/1
  adder_1_10/2(dout) -> scale_1_10/1
  convert_1_9/1 -> pol1_out9/1
  scale_1_9/1 -> convert_1_9/1
  adder_1_9/2(dout) -> scale_1_9/1
  convert_1_8/1 -> pol1_out8/1
  scale_1_8/1 -> convert_1_8/1
  adder_1_8/2(dout) -> scale_1_8/1
  convert_1_7/1 -> pol1_out7/1
  scale_1_7/1 -> convert_1_7/1
  adder_1_7/2(dout) -> scale_1_7/1
  convert_1_6/1 -> pol1_out6/1
  scale_1_6/1 -> convert_1_6/1
  adder_1_6/2(dout) -> scale_1_6/1
  convert_1_5/1 -> pol1_out5/1
  scale_1_5/1 -> convert_1_5/1
  adder_1_5/2(dout) -> scale_1_5/1
  convert_1_4/1 -> pol1_out4/1
  scale_1_4/1 -> convert_1_4/1
  adder_1_4/2(dout) -> scale_1_4/1
  convert_1_3/1 -> pol1_out3/1
  scale_1_3/1 -> convert_1_3/1
  adder_1_3/2(dout) -> scale_1_3/1
  convert_1_2/1 -> pol1_out2/1
  scale_1_2/1 -> convert_1_2/1
  adder_1_2/2(dout) -> scale_1_2/1
  scale_1_1/1 -> convert_1_1/1
  adder_1_1/1(sync_out) -> delay1/1
  pol1_in16/1 -> pol1_in16_coeffs/1(din)
  pol1_in15/1 -> pol1_in15_coeffs/1(din)
  pol1_in14/1 -> pol1_in14_coeffs/1(din)
  pol1_in13/1 -> pol1_in13_coeffs/1(din)
  pol1_in12/1 -> pol1_in12_coeffs/1(din)
  pol1_in11/1 -> pol1_in11_coeffs/1(din)
  pol1_in10/1 -> pol1_in10_coeffs/1(din)
  pol1_in9/1 -> pol1_in9_coeffs/1(din)
  pol1_in8/1 -> pol1_in8_coeffs/1(din)
  pol1_in7/1 -> pol1_in7_coeffs/1(din)
  pol1_in6/1 -> pol1_in6_coeffs/1(din)
  pol1_in5/1 -> pol1_in5_coeffs/1(din)
  pol1_in4/1 -> pol1_in4_coeffs/1(din)
  pol1_in3/1 -> pol1_in3_coeffs/1(din)
  pol1_in2/1 -> pol1_in2_coeffs/1(din)
  pol1_in1_coeffs/3(coeff) -> pol1_in1_first_tap/3(coeffs)
  pol1_in1_coeffs/2(sync_out) -> pol1_in1_first_tap/2(sync)
  sync/1 -> pol1_in16_coeffs/2(sync), pol1_in15_coeffs/2(sync), pol1_in14_coeffs/2(sync), pol1_in13_coeffs/2(sync), pol1_in12_coeffs/2(sync), pol1_in11_coeffs/2(sync), pol1_in10_coeffs/2(sync), pol1_in9_coeffs/2(sync), pol1_in8_coeffs/2(sync), pol1_in7_coeffs/2(sync), pol1_in6_coeffs/2(sync), pol1_in5_coeffs/2(sync), pol1_in4_coeffs/2(sync), pol1_in3_coeffs/2(sync), pol1_in2_coeffs/2(sync), pol1_in1_coeffs/2(sync), Delay2/1
  pol1_in1/1 -> pol1_in1_coeffs/1(din)
  pol1_in1_last_tap/1(tap_out) -> adder_1_1/5(din4)
  pol1_in1_tap1/2(sync_out) -> pol1_in1_tap4/2(sync)
  pol1_in1_first_tap1/5(add_out) -> pol1_in1_tap1/4(addr_in)
  pol1_in1_tap1/6(write_en_out) -> pol1_in1_tap4/5(write_en_in)
  pol1_in1_tap1/3(coeff_out) -> pol1_in1_tap4/3(coeff)
  pol1_in1_tap1/5(add_out) -> pol1_in1_tap4/4(addr_in)
  pol1_in1_tap1/4(taps_out) -> Delay14/1
  pol1_in1_last_tap1/2(sync_out) -> Delay12/1
  pol1_in2_coeffs/2(sync_out) -> pol1_in1_first_tap1/2(sync)
  pol1_in1_first_tap1/1(dout) -> pol1_in1_tap1/1(din)
  pol1_in2_coeffs/1(dout) -> pol1_in1_first_tap1/1(din)
  pol1_in1_tap4/2(sync_out) -> pol1_in1_last_tap1/2(sync)
  pol1_in1_first_tap1/3(coeff_out) -> pol1_in1_tap1/3(coeff)
  [tap_write_en] -> pol1_in1_first_tap1/5(write_en_in)
  [addr] -> pol1_in1_first_tap1/4(addr_in)
  pol1_in1_first_tap1/2(sync_out) -> pol1_in1_tap1/2(sync)
  pol1_in1_last_tap1/1(tap_out) -> adder_1_2/5(din4)
  pol1_in2_coeffs/3(coeff) -> pol1_in1_first_tap1/3(coeffs)
  Delay12/1 -> Delay11/1
  pol1_in1_first_tap1/6(write_en_out) -> pol1_in1_tap1/5(write_en_in)
  Delay14/1 -> adder_1_2/3(din2)
  Delay11/1 -> adder_1_2/1(sync)
  pol1_in1_tap4/4(taps_out) -> Delay15/1
  Delay13/1 -> adder_1_2/2(din1)
  pol1_in1_first_tap1/4(taps_out) -> Delay13/1
  pol1_in1_tap4/3(coeff_out) -> pol1_in1_last_tap1/3(coeff)
  pol1_in1_tap1/1(dout) -> pol1_in1_tap4/1(din)
  pol1_in1_tap4/1(dout) -> pol1_in1_last_tap1/1(din)
  Delay15/1 -> adder_1_2/4(din3)
  pol1_in1_tap5/2(sync_out) -> pol1_in1_tap6/2(sync)
  pol1_in1_first_tap2/5(add_out) -> pol1_in1_tap5/4(addr_in)
  pol1_in1_tap5/6(write_en_out) -> pol1_in1_tap6/5(write_en_in)
  pol1_in1_tap5/3(coeff_out) -> pol1_in1_tap6/3(coeff)
  pol1_in1_tap5/5(add_out) -> pol1_in1_tap6/4(addr_in)
  pol1_in1_tap5/4(taps_out) -> Delay19/1
  pol1_in1_last_tap2/2(sync_out) -> Delay17/1
  pol1_in3_coeffs/2(sync_out) -> pol1_in1_first_tap2/2(sync)
  pol1_in1_first_tap2/1(dout) -> pol1_in1_tap5/1(din)
  pol1_in3_coeffs/1(dout) -> pol1_in1_first_tap2/1(din)
  pol1_in1_tap6/2(sync_out) -> pol1_in1_last_tap2/2(sync)
  pol1_in1_first_tap2/3(coeff_out) -> pol1_in1_tap5/3(coeff)
  [tap_write_en] -> pol1_in1_first_tap2/5(write_en_in)
  [addr] -> pol1_in1_first_tap2/4(addr_in)
  pol1_in1_first_tap2/2(sync_out) -> pol1_in1_tap5/2(sync)
  pol1_in1_last_tap2/1(tap_out) -> adder_1_3/5(din4)
  pol1_in3_coeffs/3(coeff) -> pol1_in1_first_tap2/3(coeffs)
  Delay17/1 -> Delay16/1
  pol1_in1_first_tap2/6(write_en_out) -> pol1_in1_tap5/5(write_en_in)
  Delay19/1 -> adder_1_3/3(din2)
  Delay16/1 -> adder_1_3/1(sync)
  pol1_in1_tap6/4(taps_out) -> Delay20/1
  Delay18/1 -> adder_1_3/2(din1)
  pol1_in1_first_tap2/4(taps_out) -> Delay18/1
  pol1_in1_tap6/3(coeff_out) -> pol1_in1_last_tap2/3(coeff)
  pol1_in1_tap5/1(dout) -> pol1_in1_tap6/1(din)
  pol1_in1_tap6/1(dout) -> pol1_in1_last_tap2/1(din)
  Delay20/1 -> adder_1_3/4(din3)
  pol1_in1_tap7/2(sync_out) -> pol1_in1_tap8/2(sync)
  pol1_in1_first_tap3/5(add_out) -> pol1_in1_tap7/4(addr_in)
  pol1_in1_tap7/6(write_en_out) -> pol1_in1_tap8/5(write_en_in)
  pol1_in1_tap7/3(coeff_out) -> pol1_in1_tap8/3(coeff)
  pol1_in1_tap7/5(add_out) -> pol1_in1_tap8/4(addr_in)
  pol1_in1_tap7/4(taps_out) -> Delay24/1
  pol1_in1_last_tap3/2(sync_out) -> Delay22/1
  pol1_in4_coeffs/2(sync_out) -> pol1_in1_first_tap3/2(sync)
  pol1_in1_first_tap3/1(dout) -> pol1_in1_tap7/1(din)
  pol1_in4_coeffs/1(dout) -> pol1_in1_first_tap3/1(din)
  pol1_in1_tap8/2(sync_out) -> pol1_in1_last_tap3/2(sync)
  pol1_in1_first_tap3/3(coeff_out) -> pol1_in1_tap7/3(coeff)
  [tap_write_en] -> pol1_in1_first_tap3/5(write_en_in)
  [addr] -> pol1_in1_first_tap3/4(addr_in)
  pol1_in1_first_tap3/2(sync_out) -> pol1_in1_tap7/2(sync)
  pol1_in1_last_tap3/1(tap_out) -> adder_1_4/5(din4)
  pol1_in4_coeffs/3(coeff) -> pol1_in1_first_tap3/3(coeffs)
  Delay22/1 -> Delay21/1
  pol1_in1_first_tap3/6(write_en_out) -> pol1_in1_tap7/5(write_en_in)
  Delay24/1 -> adder_1_4/3(din2)
  Delay21/1 -> adder_1_4/1(sync)
  pol1_in1_tap8/4(taps_out) -> Delay25/1
  Delay23/1 -> adder_1_4/2(din1)
  pol1_in1_first_tap3/4(taps_out) -> Delay23/1
  pol1_in1_tap8/3(coeff_out) -> pol1_in1_last_tap3/3(coeff)
  pol1_in1_tap7/1(dout) -> pol1_in1_tap8/1(din)
  pol1_in1_tap8/1(dout) -> pol1_in1_last_tap3/1(din)
  Delay25/1 -> adder_1_4/4(din3)
  pol1_in1_tap9/2(sync_out) -> pol1_in1_tap10/2(sync)
  pol1_in1_first_tap4/5(add_out) -> pol1_in1_tap9/4(addr_in)
  pol1_in1_tap9/6(write_en_out) -> pol1_in1_tap10/5(write_en_in)
  pol1_in1_tap9/3(coeff_out) -> pol1_in1_tap10/3(coeff)
  pol1_in1_tap9/5(add_out) -> pol1_in1_tap10/4(addr_in)
  pol1_in1_tap9/4(taps_out) -> Delay29/1
  pol1_in1_last_tap4/2(sync_out) -> Delay27/1
  pol1_in5_coeffs/2(sync_out) -> pol1_in1_first_tap4/2(sync)
  pol1_in1_first_tap4/1(dout) -> pol1_in1_tap9/1(din)
  pol1_in5_coeffs/1(dout) -> pol1_in1_first_tap4/1(din)
  pol1_in1_tap10/2(sync_out) -> pol1_in1_last_tap4/2(sync)
  pol1_in1_first_tap4/3(coeff_out) -> pol1_in1_tap9/3(coeff)
  [tap_write_en] -> pol1_in1_first_tap4/5(write_en_in)
  [addr] -> pol1_in1_first_tap4/4(addr_in)
  pol1_in1_first_tap4/2(sync_out) -> pol1_in1_tap9/2(sync)
  pol1_in1_last_tap4/1(tap_out) -> adder_1_5/5(din4)
  pol1_in5_coeffs/3(coeff) -> pol1_in1_first_tap4/3(coeffs)
  Delay27/1 -> Delay26/1
  pol1_in1_first_tap4/6(write_en_out) -> pol1_in1_tap9/5(write_en_in)
  Delay29/1 -> adder_1_5/3(din2)
  Delay26/1 -> adder_1_5/1(sync)
  pol1_in1_tap10/4(taps_out) -> Delay30/1
  Delay28/1 -> adder_1_5/2(din1)
  pol1_in1_first_tap4/4(taps_out) -> Delay28/1
  pol1_in1_tap10/3(coeff_out) -> pol1_in1_last_tap4/3(coeff)
  pol1_in1_tap9/1(dout) -> pol1_in1_tap10/1(din)
  pol1_in1_tap10/1(dout) -> pol1_in1_last_tap4/1(din)
  Delay30/1 -> adder_1_5/4(din3)
  pol1_in1_tap11/2(sync_out) -> pol1_in1_tap12/2(sync)
  pol1_in1_first_tap5/5(add_out) -> pol1_in1_tap11/4(addr_in)
  pol1_in1_tap11/6(write_en_out) -> pol1_in1_tap12/5(write_en_in)
  pol1_in1_tap11/3(coeff_out) -> pol1_in1_tap12/3(coeff)
  pol1_in1_tap11/5(add_out) -> pol1_in1_tap12/4(addr_in)
  pol1_in1_tap11/4(taps_out) -> Delay34/1
  pol1_in1_last_tap5/2(sync_out) -> Delay32/1
  pol1_in6_coeffs/2(sync_out) -> pol1_in1_first_tap5/2(sync)
  pol1_in1_first_tap5/1(dout) -> pol1_in1_tap11/1(din)
  pol1_in6_coeffs/1(dout) -> pol1_in1_first_tap5/1(din)
  pol1_in1_tap12/2(sync_out) -> pol1_in1_last_tap5/2(sync)
  pol1_in1_first_tap5/3(coeff_out) -> pol1_in1_tap11/3(coeff)
  [tap_write_en] -> pol1_in1_first_tap5/5(write_en_in)
  [addr] -> pol1_in1_first_tap5/4(addr_in)
  pol1_in1_first_tap5/2(sync_out) -> pol1_in1_tap11/2(sync)
  pol1_in1_last_tap5/1(tap_out) -> adder_1_6/5(din4)
  pol1_in6_coeffs/3(coeff) -> pol1_in1_first_tap5/3(coeffs)
  Delay32/1 -> Delay31/1
  pol1_in1_first_tap5/6(write_en_out) -> pol1_in1_tap11/5(write_en_in)
  Delay34/1 -> adder_1_6/3(din2)
  Delay31/1 -> adder_1_6/1(sync)
  pol1_in1_tap12/4(taps_out) -> Delay35/1
  Delay33/1 -> adder_1_6/2(din1)
  pol1_in1_first_tap5/4(taps_out) -> Delay33/1
  pol1_in1_tap12/3(coeff_out) -> pol1_in1_last_tap5/3(coeff)
  pol1_in1_tap11/1(dout) -> pol1_in1_tap12/1(din)
  pol1_in1_tap12/1(dout) -> pol1_in1_last_tap5/1(din)
  Delay35/1 -> adder_1_6/4(din3)
  pol1_in1_tap13/2(sync_out) -> pol1_in1_tap14/2(sync)
  pol1_in1_first_tap6/5(add_out) -> pol1_in1_tap13/4(addr_in)
  pol1_in1_tap13/6(write_en_out) -> pol1_in1_tap14/5(write_en_in)
  pol1_in1_tap13/3(coeff_out) -> pol1_in1_tap14/3(coeff)
  pol1_in1_tap13/5(add_out) -> pol1_in1_tap14/4(addr_in)
  pol1_in1_tap13/4(taps_out) -> Delay39/1
  pol1_in1_last_tap6/2(sync_out) -> Delay37/1
  pol1_in7_coeffs/2(sync_out) -> pol1_in1_first_tap6/2(sync)
  pol1_in1_first_tap6/1(dout) -> pol1_in1_tap13/1(din)
  pol1_in7_coeffs/1(dout) -> pol1_in1_first_tap6/1(din)
  pol1_in1_tap14/2(sync_out) -> pol1_in1_last_tap6/2(sync)
  pol1_in1_first_tap6/3(coeff_out) -> pol1_in1_tap13/3(coeff)
  [tap_write_en] -> pol1_in1_first_tap6/5(write_en_in)
  [addr] -> pol1_in1_first_tap6/4(addr_in)
  pol1_in1_first_tap6/2(sync_out) -> pol1_in1_tap13/2(sync)
  pol1_in1_last_tap6/1(tap_out) -> adder_1_7/5(din4)
  pol1_in7_coeffs/3(coeff) -> pol1_in1_first_tap6/3(coeffs)
  Delay37/1 -> Delay36/1
  pol1_in1_first_tap6/6(write_en_out) -> pol1_in1_tap13/5(write_en_in)
  Delay39/1 -> adder_1_7/3(din2)
  Delay36/1 -> adder_1_7/1(sync)
  pol1_in1_tap14/4(taps_out) -> Delay40/1
  Delay38/1 -> adder_1_7/2(din1)
  pol1_in1_first_tap6/4(taps_out) -> Delay38/1
  pol1_in1_tap14/3(coeff_out) -> pol1_in1_last_tap6/3(coeff)
  pol1_in1_tap13/1(dout) -> pol1_in1_tap14/1(din)
  pol1_in1_tap14/1(dout) -> pol1_in1_last_tap6/1(din)
  Delay40/1 -> adder_1_7/4(din3)
  pol1_in1_tap15/2(sync_out) -> pol1_in1_tap16/2(sync)
  pol1_in1_first_tap7/5(add_out) -> pol1_in1_tap15/4(addr_in)
  pol1_in1_tap15/6(write_en_out) -> pol1_in1_tap16/5(write_en_in)
  pol1_in1_tap15/3(coeff_out) -> pol1_in1_tap16/3(coeff)
  pol1_in1_tap15/5(add_out) -> pol1_in1_tap16/4(addr_in)
  pol1_in1_tap15/4(taps_out) -> Delay44/1
  pol1_in1_last_tap7/2(sync_out) -> Delay42/1
  pol1_in8_coeffs/2(sync_out) -> pol1_in1_first_tap7/2(sync)
  pol1_in1_first_tap7/1(dout) -> pol1_in1_tap15/1(din)
  pol1_in8_coeffs/1(dout) -> pol1_in1_first_tap7/1(din)
  pol1_in1_tap16/2(sync_out) -> pol1_in1_last_tap7/2(sync)
  pol1_in1_first_tap7/3(coeff_out) -> pol1_in1_tap15/3(coeff)
  [tap_write_en] -> pol1_in1_first_tap7/5(write_en_in)
  [addr] -> pol1_in1_first_tap7/4(addr_in)
  pol1_in1_first_tap7/2(sync_out) -> pol1_in1_tap15/2(sync)
  pol1_in1_last_tap7/1(tap_out) -> adder_1_8/5(din4)
  pol1_in8_coeffs/3(coeff) -> pol1_in1_first_tap7/3(coeffs)
  Delay42/1 -> Delay41/1
  pol1_in1_first_tap7/6(write_en_out) -> pol1_in1_tap15/5(write_en_in)
  Delay44/1 -> adder_1_8/3(din2)
  Delay41/1 -> adder_1_8/1(sync)
  pol1_in1_tap16/4(taps_out) -> Delay45/1
  Delay43/1 -> adder_1_8/2(din1)
  pol1_in1_first_tap7/4(taps_out) -> Delay43/1
  pol1_in1_tap16/3(coeff_out) -> pol1_in1_last_tap7/3(coeff)
  pol1_in1_tap15/1(dout) -> pol1_in1_tap16/1(din)
  pol1_in1_tap16/1(dout) -> pol1_in1_last_tap7/1(din)
  Delay45/1 -> adder_1_8/4(din3)
  pol1_in1_tap17/2(sync_out) -> pol1_in1_tap18/2(sync)
  pol1_in1_first_tap8/5(add_out) -> pol1_in1_tap17/4(addr_in)
  pol1_in1_tap17/6(write_en_out) -> pol1_in1_tap18/5(write_en_in)
  pol1_in1_tap17/3(coeff_out) -> pol1_in1_tap18/3(coeff)
  pol1_in1_tap17/5(add_out) -> pol1_in1_tap18/4(addr_in)
  pol1_in1_tap17/4(taps_out) -> Delay49/1
  pol1_in1_last_tap8/2(sync_out) -> Delay47/1
  pol1_in9_coeffs/2(sync_out) -> pol1_in1_first_tap8/2(sync)
  pol1_in1_first_tap8/1(dout) -> pol1_in1_tap17/1(din)
  pol1_in9_coeffs/1(dout) -> pol1_in1_first_tap8/1(din)
  pol1_in1_tap18/2(sync_out) -> pol1_in1_last_tap8/2(sync)
  pol1_in1_first_tap8/3(coeff_out) -> pol1_in1_tap17/3(coeff)
  [tap_write_en] -> pol1_in1_first_tap8/5(write_en_in)
  [addr] -> pol1_in1_first_tap8/4(addr_in)
  pol1_in1_first_tap8/2(sync_out) -> pol1_in1_tap17/2(sync)
  pol1_in1_last_tap8/1(tap_out) -> adder_1_9/5(din4)
  pol1_in9_coeffs/3(coeff) -> pol1_in1_first_tap8/3(coeffs)
  Delay47/1 -> Delay46/1
  pol1_in1_first_tap8/6(write_en_out) -> pol1_in1_tap17/5(write_en_in)
  Delay49/1 -> adder_1_9/3(din2)
  Delay46/1 -> adder_1_9/1(sync)
  pol1_in1_tap18/4(taps_out) -> Delay50/1
  Delay48/1 -> adder_1_9/2(din1)
  pol1_in1_first_tap8/4(taps_out) -> Delay48/1
  pol1_in1_tap18/3(coeff_out) -> pol1_in1_last_tap8/3(coeff)
  pol1_in1_tap17/1(dout) -> pol1_in1_tap18/1(din)
  pol1_in1_tap18/1(dout) -> pol1_in1_last_tap8/1(din)
  Delay50/1 -> adder_1_9/4(din3)
  pol1_in1_tap19/2(sync_out) -> pol1_in1_tap20/2(sync)
  pol1_in1_first_tap9/5(add_out) -> pol1_in1_tap19/4(addr_in)
  pol1_in1_tap19/6(write_en_out) -> pol1_in1_tap20/5(write_en_in)
  pol1_in1_tap19/3(coeff_out) -> pol1_in1_tap20/3(coeff)
  pol1_in1_tap19/5(add_out) -> pol1_in1_tap20/4(addr_in)
  pol1_in1_tap19/4(taps_out) -> Delay54/1
  pol1_in1_last_tap9/2(sync_out) -> Delay52/1
  pol1_in10_coeffs/2(sync_out) -> pol1_in1_first_tap9/2(sync)
  pol1_in1_first_tap9/1(dout) -> pol1_in1_tap19/1(din)
  pol1_in10_coeffs/1(dout) -> pol1_in1_first_tap9/1(din)
  pol1_in1_tap20/2(sync_out) -> pol1_in1_last_tap9/2(sync)
  pol1_in1_first_tap9/3(coeff_out) -> pol1_in1_tap19/3(coeff)
  [tap_write_en] -> pol1_in1_first_tap9/5(write_en_in)
  [addr] -> pol1_in1_first_tap9/4(addr_in)
  pol1_in1_first_tap9/2(sync_out) -> pol1_in1_tap19/2(sync)
  pol1_in1_last_tap9/1(tap_out) -> adder_1_10/5(din4)
  pol1_in10_coeffs/3(coeff) -> pol1_in1_first_tap9/3(coeffs)
  Delay52/1 -> Delay51/1
  pol1_in1_first_tap9/6(write_en_out) -> pol1_in1_tap19/5(write_en_in)
  Delay54/1 -> adder_1_10/3(din2)
  Delay51/1 -> adder_1_10/1(sync)
  pol1_in1_tap20/4(taps_out) -> Delay55/1
  Delay53/1 -> adder_1_10/2(din1)
  pol1_in1_first_tap9/4(taps_out) -> Delay53/1
  pol1_in1_tap20/3(coeff_out) -> pol1_in1_last_tap9/3(coeff)
  pol1_in1_tap19/1(dout) -> pol1_in1_tap20/1(din)
  pol1_in1_tap20/1(dout) -> pol1_in1_last_tap9/1(din)
  Delay55/1 -> adder_1_10/4(din3)
  pol1_in1_tap21/2(sync_out) -> pol1_in1_tap22/2(sync)
  pol1_in1_first_tap10/5(add_out) -> pol1_in1_tap21/4(addr_in)
  pol1_in1_tap21/6(write_en_out) -> pol1_in1_tap22/5(write_en_in)
  pol1_in1_tap21/3(coeff_out) -> pol1_in1_tap22/3(coeff)
  pol1_in1_tap21/5(add_out) -> pol1_in1_tap22/4(addr_in)
  pol1_in1_tap21/4(taps_out) -> Delay59/1
  pol1_in1_last_tap10/2(sync_out) -> Delay57/1
  pol1_in11_coeffs/2(sync_out) -> pol1_in1_first_tap10/2(sync)
  pol1_in1_first_tap10/1(dout) -> pol1_in1_tap21/1(din)
  pol1_in11_coeffs/1(dout) -> pol1_in1_first_tap10/1(din)
  pol1_in1_tap22/2(sync_out) -> pol1_in1_last_tap10/2(sync)
  pol1_in1_first_tap10/3(coeff_out) -> pol1_in1_tap21/3(coeff)
  [tap_write_en] -> pol1_in1_first_tap10/5(write_en_in)
  [addr] -> pol1_in1_first_tap10/4(addr_in)
  pol1_in1_first_tap10/2(sync_out) -> pol1_in1_tap21/2(sync)
  pol1_in1_last_tap10/1(tap_out) -> adder_1_11/5(din4)
  pol1_in11_coeffs/3(coeff) -> pol1_in1_first_tap10/3(coeffs)
  Delay57/1 -> Delay56/1
  pol1_in1_first_tap10/6(write_en_out) -> pol1_in1_tap21/5(write_en_in)
  Delay59/1 -> adder_1_11/3(din2)
  Delay56/1 -> adder_1_11/1(sync)
  pol1_in1_tap22/4(taps_out) -> Delay60/1
  Delay58/1 -> adder_1_11/2(din1)
  pol1_in1_first_tap10/4(taps_out) -> Delay58/1
  pol1_in1_tap22/3(coeff_out) -> pol1_in1_last_tap10/3(coeff)
  pol1_in1_tap21/1(dout) -> pol1_in1_tap22/1(din)
  pol1_in1_tap22/1(dout) -> pol1_in1_last_tap10/1(din)
  Delay60/1 -> adder_1_11/4(din3)
  pol1_in1_tap23/2(sync_out) -> pol1_in1_tap24/2(sync)
  pol1_in1_first_tap11/5(add_out) -> pol1_in1_tap23/4(addr_in)
  pol1_in1_tap23/6(write_en_out) -> pol1_in1_tap24/5(write_en_in)
  pol1_in1_tap23/3(coeff_out) -> pol1_in1_tap24/3(coeff)
  pol1_in1_tap23/5(add_out) -> pol1_in1_tap24/4(addr_in)
  pol1_in1_tap23/4(taps_out) -> Delay64/1
  pol1_in1_last_tap11/2(sync_out) -> Delay62/1
  pol1_in12_coeffs/2(sync_out) -> pol1_in1_first_tap11/2(sync)
  pol1_in1_first_tap11/1(dout) -> pol1_in1_tap23/1(din)
  pol1_in12_coeffs/1(dout) -> pol1_in1_first_tap11/1(din)
  pol1_in1_tap24/2(sync_out) -> pol1_in1_last_tap11/2(sync)
  pol1_in1_first_tap11/3(coeff_out) -> pol1_in1_tap23/3(coeff)
  [tap_write_en] -> pol1_in1_first_tap11/5(write_en_in)
  [addr] -> pol1_in1_first_tap11/4(addr_in)
  pol1_in1_first_tap11/2(sync_out) -> pol1_in1_tap23/2(sync)
  pol1_in1_last_tap11/1(tap_out) -> adder_1_12/5(din4)
  pol1_in12_coeffs/3(coeff) -> pol1_in1_first_tap11/3(coeffs)
  Delay62/1 -> Delay61/1
  pol1_in1_first_tap11/6(write_en_out) -> pol1_in1_tap23/5(write_en_in)
  Delay64/1 -> adder_1_12/3(din2)
  Delay61/1 -> adder_1_12/1(sync)
  pol1_in1_tap24/4(taps_out) -> Delay65/1
  Delay63/1 -> adder_1_12/2(din1)
  pol1_in1_first_tap11/4(taps_out) -> Delay63/1
  pol1_in1_tap24/3(coeff_out) -> pol1_in1_last_tap11/3(coeff)
  pol1_in1_tap23/1(dout) -> pol1_in1_tap24/1(din)
  pol1_in1_tap24/1(dout) -> pol1_in1_last_tap11/1(din)
  Delay65/1 -> adder_1_12/4(din3)
  pol1_in1_tap25/2(sync_out) -> pol1_in1_tap26/2(sync)
  pol1_in1_first_tap12/5(add_out) -> pol1_in1_tap25/4(addr_in)
  pol1_in1_tap25/6(write_en_out) -> pol1_in1_tap26/5(write_en_in)
  pol1_in1_tap25/3(coeff_out) -> pol1_in1_tap26/3(coeff)
  pol1_in1_tap25/5(add_out) -> pol1_in1_tap26/4(addr_in)
  pol1_in1_tap25/4(taps_out) -> Delay69/1
  pol1_in1_last_tap12/2(sync_out) -> Delay67/1
  pol1_in13_coeffs/2(sync_out) -> pol1_in1_first_tap12/2(sync)
  pol1_in1_first_tap12/1(dout) -> pol1_in1_tap25/1(din)
  pol1_in13_coeffs/1(dout) -> pol1_in1_first_tap12/1(din)
  pol1_in1_tap26/2(sync_out) -> pol1_in1_last_tap12/2(sync)
  pol1_in1_first_tap12/3(coeff_out) -> pol1_in1_tap25/3(coeff)
  [tap_write_en] -> pol1_in1_first_tap12/5(write_en_in)
  [addr] -> pol1_in1_first_tap12/4(addr_in)
  pol1_in1_first_tap12/2(sync_out) -> pol1_in1_tap25/2(sync)
  pol1_in1_last_tap12/1(tap_out) -> adder_1_13/5(din4)
  pol1_in13_coeffs/3(coeff) -> pol1_in1_first_tap12/3(coeffs)
  Delay67/1 -> Delay66/1
  pol1_in1_first_tap12/6(write_en_out) -> pol1_in1_tap25/5(write_en_in)
  Delay69/1 -> adder_1_13/3(din2)
  Delay66/1 -> adder_1_13/1(sync)
  pol1_in1_tap26/4(taps_out) -> Delay70/1
  Delay68/1 -> adder_1_13/2(din1)
  pol1_in1_first_tap12/4(taps_out) -> Delay68/1
  pol1_in1_tap26/3(coeff_out) -> pol1_in1_last_tap12/3(coeff)
  pol1_in1_tap25/1(dout) -> pol1_in1_tap26/1(din)
  pol1_in1_tap26/1(dout) -> pol1_in1_last_tap12/1(din)
  Delay70/1 -> adder_1_13/4(din3)
  pol1_in1_tap27/2(sync_out) -> pol1_in1_tap28/2(sync)
  pol1_in1_first_tap13/5(add_out) -> pol1_in1_tap27/4(addr_in)
  pol1_in1_tap27/6(write_en_out) -> pol1_in1_tap28/5(write_en_in)
  pol1_in1_tap27/3(coeff_out) -> pol1_in1_tap28/3(coeff)
  pol1_in1_tap27/5(add_out) -> pol1_in1_tap28/4(addr_in)
  pol1_in1_tap27/4(taps_out) -> Delay74/1
  pol1_in1_last_tap13/2(sync_out) -> Delay72/1
  pol1_in14_coeffs/2(sync_out) -> pol1_in1_first_tap13/2(sync)
  pol1_in1_first_tap13/1(dout) -> pol1_in1_tap27/1(din)
  pol1_in14_coeffs/1(dout) -> pol1_in1_first_tap13/1(din)
  pol1_in1_tap28/2(sync_out) -> pol1_in1_last_tap13/2(sync)
  pol1_in1_first_tap13/3(coeff_out) -> pol1_in1_tap27/3(coeff)
  [tap_write_en] -> pol1_in1_first_tap13/5(write_en_in)
  [addr] -> pol1_in1_first_tap13/4(addr_in)
  pol1_in1_first_tap13/2(sync_out) -> pol1_in1_tap27/2(sync)
  pol1_in1_last_tap13/1(tap_out) -> adder_1_14/5(din4)
  pol1_in14_coeffs/3(coeff) -> pol1_in1_first_tap13/3(coeffs)
  Delay72/1 -> Delay71/1
  pol1_in1_first_tap13/6(write_en_out) -> pol1_in1_tap27/5(write_en_in)
  Delay74/1 -> adder_1_14/3(din2)
  Delay71/1 -> adder_1_14/1(sync)
  pol1_in1_tap28/4(taps_out) -> Delay75/1
  Delay73/1 -> adder_1_14/2(din1)
  pol1_in1_first_tap13/4(taps_out) -> Delay73/1
  pol1_in1_tap28/3(coeff_out) -> pol1_in1_last_tap13/3(coeff)
  pol1_in1_tap27/1(dout) -> pol1_in1_tap28/1(din)
  pol1_in1_tap28/1(dout) -> pol1_in1_last_tap13/1(din)
  Delay75/1 -> adder_1_14/4(din3)
  pol1_in1_tap29/2(sync_out) -> pol1_in1_tap30/2(sync)
  pol1_in1_first_tap14/5(add_out) -> pol1_in1_tap29/4(addr_in)
  pol1_in1_tap29/6(write_en_out) -> pol1_in1_tap30/5(write_en_in)
  pol1_in1_tap29/3(coeff_out) -> pol1_in1_tap30/3(coeff)
  pol1_in1_tap29/5(add_out) -> pol1_in1_tap30/4(addr_in)
  pol1_in1_tap29/4(taps_out) -> Delay80/1
  pol1_in1_last_tap14/2(sync_out) -> Delay78/1
  pol1_in15_coeffs/2(sync_out) -> pol1_in1_first_tap14/2(sync)
  pol1_in1_first_tap14/1(dout) -> pol1_in1_tap29/1(din)
  pol1_in15_coeffs/1(dout) -> pol1_in1_first_tap14/1(din)
  pol1_in1_tap30/2(sync_out) -> pol1_in1_last_tap14/2(sync)
  pol1_in1_first_tap14/3(coeff_out) -> pol1_in1_tap29/3(coeff)
  [tap_write_en] -> pol1_in1_first_tap14/5(write_en_in)
  [addr] -> pol1_in1_first_tap14/4(addr_in)
  pol1_in1_first_tap14/2(sync_out) -> pol1_in1_tap29/2(sync)
  pol1_in1_last_tap14/1(tap_out) -> adder_1_15/5(din4)
  pol1_in15_coeffs/3(coeff) -> pol1_in1_first_tap14/3(coeffs)
  Delay78/1 -> Delay77/1
  pol1_in1_first_tap14/6(write_en_out) -> pol1_in1_tap29/5(write_en_in)
  Delay80/1 -> adder_1_15/3(din2)
  Delay77/1 -> adder_1_15/1(sync)
  pol1_in1_tap30/4(taps_out) -> Delay81/1
  Delay79/1 -> adder_1_15/2(din1)
  pol1_in1_first_tap14/4(taps_out) -> Delay79/1
  pol1_in1_tap30/3(coeff_out) -> pol1_in1_last_tap14/3(coeff)
  pol1_in1_tap29/1(dout) -> pol1_in1_tap30/1(din)
  pol1_in1_tap30/1(dout) -> pol1_in1_last_tap14/1(din)
  Delay81/1 -> adder_1_15/4(din3)
  pol1_in1_tap31/2(sync_out) -> pol1_in1_tap32/2(sync)
  pol1_in1_first_tap15/5(add_out) -> pol1_in1_tap31/4(addr_in)
  pol1_in1_tap31/6(write_en_out) -> pol1_in1_tap32/5(write_en_in)
  pol1_in1_tap31/3(coeff_out) -> pol1_in1_tap32/3(coeff)
  pol1_in1_tap31/5(add_out) -> pol1_in1_tap32/4(addr_in)
  pol1_in1_tap31/4(taps_out) -> Delay85/1
  pol1_in1_last_tap15/2(sync_out) -> Delay83/1
  pol1_in16_coeffs/2(sync_out) -> pol1_in1_first_tap15/2(sync)
  pol1_in1_first_tap15/1(dout) -> pol1_in1_tap31/1(din)
  pol1_in16_coeffs/1(dout) -> pol1_in1_first_tap15/1(din)
  pol1_in1_tap32/2(sync_out) -> pol1_in1_last_tap15/2(sync)
  pol1_in1_first_tap15/3(coeff_out) -> pol1_in1_tap31/3(coeff)
  [tap_write_en] -> pol1_in1_first_tap15/5(write_en_in)
  [addr] -> pol1_in1_first_tap15/4(addr_in)
  pol1_in1_first_tap15/2(sync_out) -> pol1_in1_tap31/2(sync)
  pol1_in1_last_tap15/1(tap_out) -> adder_1_16/5(din4)
  pol1_in16_coeffs/3(coeff) -> pol1_in1_first_tap15/3(coeffs)
  Delay83/1 -> Delay82/1
  pol1_in1_first_tap15/6(write_en_out) -> pol1_in1_tap31/5(write_en_in)
  Delay85/1 -> adder_1_16/3(din2)
  Delay82/1 -> adder_1_16/1(sync)
  pol1_in1_tap32/4(taps_out) -> Delay86/1
  Delay84/1 -> adder_1_16/2(din1)
  pol1_in1_first_tap15/4(taps_out) -> Delay84/1
  pol1_in1_tap32/3(coeff_out) -> pol1_in1_last_tap15/3(coeff)
  pol1_in1_tap31/1(dout) -> pol1_in1_tap32/1(din)
  pol1_in1_tap32/1(dout) -> pol1_in1_last_tap15/1(din)
  Delay86/1 -> adder_1_16/4(din3)
